simulink model "BimanualCarvingModifiedOldEMG"  (R2013a)
settings: Solver=ode4  SolverMode=SingleTasking  StartTime=0.0  StopTime=inf  FixedStep=0.0005  RelTol=1e-3
StartFcn:
  |  warndlg('Dexterit-E models cannot run under simulation. Please compile your model and run it from within Dexterit-E.');set_param(bdroot,'SimulationCommand','stop')
model workspace (MAT data in the model file):
  BKIN_STEP_TIME = 0.0005
  col_x = 1
  col_y = 2
  WIDTH = 3
  HEIGHT = 4
  TARGET_COL = 1
  LOAD = 2
  TRAJ_DURATION_COL = 3
  MAX_LOAD = 2
  FORCE_ON = 1
  HAND_RADIUS = 6
  REST_COL = 4
  TRAINING_COL = 5
  HAND_COLOR = 5
  TARGET_STROKE = 8
  TARGET_RADIUS = 9
  xMaxCursor = 15
  yMaxCursor = 16
  TARGET_COLOR = 7
  START_X = 10
  START_Y = 11
  STIFFNESS_MATERIAL = 3
  MATERIAL_MASS = 4
  MATERIAL_DAMPING = 5
  STIFFNESS_HANDS = 6
  MATERIAL_GOAL_COLOR = 12
  SCALE_VIBRATION = 7
  STONE_WIDTH = 6
  MATERIAL_DUCTILITY = 8
  TARG_COLOR = 1
  TEXT_COLOR = 13
  TEXTBOX_WIDTH = 14
  TEXTBOX_HEIGHT = 15
  ROTATION = 16
  LABEL_TEXT = 17
  LABEL_COLOR = 18
  LABEL_HEIGHT = 19
  ADVANCE_EMG_PLACEMENT = 2
  ADVANCE_EMG_MAX = 3
  EMG_ADVANCE_BUTTON = 1
  EMG_MVC_BUTTON = 2
  START_TRIAL = 3
  END_TRIAL = 4
  MUSC_NUM = 2
  HAND_DISTANCE = 3
  SYN_NUM = 4
undefined symbols (not defined in the file or in its folder): slselsubs
libraries: xpclib x9, simulink x6, General x3, KINARM_loads x2, Video x2, KINARM_IO x1, KINARM_EP_loads x1
(part 1 of 6)
CloseFcn:
  | rtwprivate ssgencode ModelCloseRequest b2lab2d
settings Model: ModifiedComment=chris -- Wed Feb 16 09:18:30 2005 -- Version 1.1384  ModifiedHistory=Feb 16/05 - Add error repeat, add offset ramp  ExtModeArmWhenConnect=off  ExtModeLogAll=off  BufferReuse=off  Creator=Chris Grebeldinger  LastModifiedBy=BKIN TECHNOLOGIES
settings DataIOCC: LimitDataPoints=off  SignalLoggingSaveFormat=ModelDataLogs  SaveOutput=off  SaveTime=off  SignalLoggingName=sigsOut
settings OptimizationCC: BlockReduction=off  BooleanDataType=off  OptimizeBlockIOStorage=off  BufferReuse=off  ExpressionFolding=off  ExpressionDepthLimit=2147483647  FoldNonRolledExpr=off  LocalBlockOutputs=off  InitFltsAndDblsToZero=on
settings DebuggingCC: SaveWithParameterizedLinksMsg=none  SignalResolutionControl=TryResolveAllWithWarning  SolverPrmCheckMsg=none  MultiTaskDSMMsg=warning  MultiTaskCondExecSysMsg=none  FcnCallInpInsideContextMsg=UseLocalSettings  StrictBusMsg=None
settings HardwareCC: ProdIntDivRoundTo=Zero  ProdEndianess=LittleEndian  ProdHWDeviceType=Generic->32-bit x86 compatible  TargetHWDeviceType=32-bit Generic
settings SFSimCC: SimParseCustomCode=off
settings RTWCC: SystemTargetFile=xpctarget.tlc  TemplateMakefile=xpc_default_tmf  Description=xPC Target  ProcessScript=xpctarget_make_rtw_hook  IncludeERTFirstTime=on  RTWCompilerOptimization=On
settings CodeAppCC: MaxIdLength=63
settings xpcTargetCC: TargetFcnLib=ansi_tfl_tmw.mat  CodeReplacementLibrary=XPC_BLAS  ParMdlRefBuildCompliant=on  ConcurrentExecutionCompliant=on  CombineSignalStateStructs=off  MATLABClassNameForMDSCustomization=xpcAperiodicCustomization  GRTInterface=on  GenerateAllocFcn=off  xPCTaskExecutionProfile=off  xPCRL32EventNumber=5000  xPCisDownloadable=off  xPCLoadParamSetFile=off  xPCConcurrentTasks=off  xPCEnableSFAnimation=off

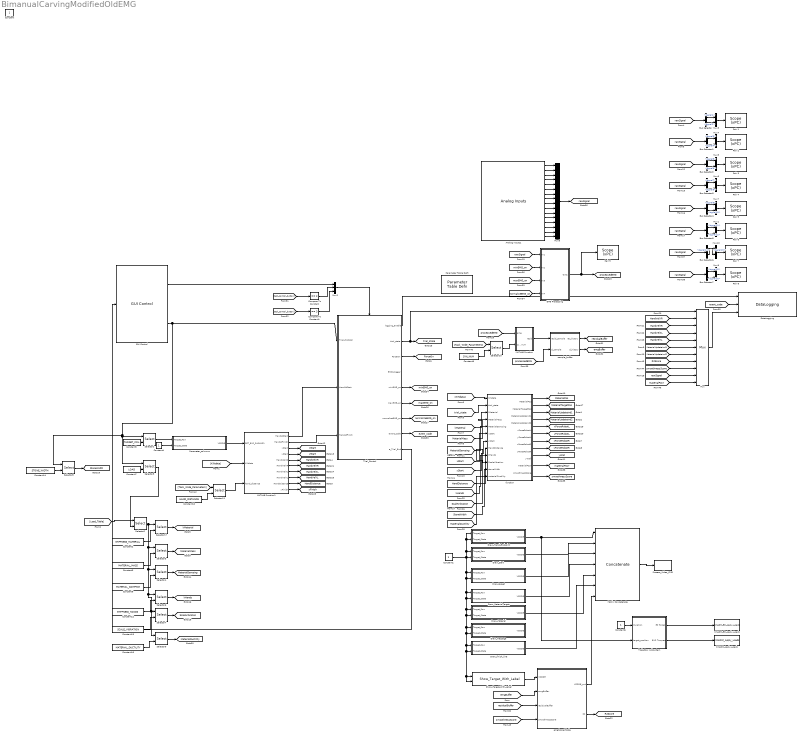
== system BimanualCarvingModifiedOldEMG ==
  Analog Inputs1 : KINARM_IO/Analog Inputs  channel=[1,2,3,4,5,6,7,8,9,10,11,12,13,14,15,16]  range=[5]  coupling=[0]  scantime6071e=1.28e-5  scantime6229=5e-6  sampletime=0.001  slot=-1  oscantime6071e=0
  Bus Selector : BusSelector  OutputSignals=signal1,signal2
  Bus Selector1 : BusSelector  OutputSignals=signal3,signal4
  Bus Selector2 : BusSelector  OutputSignals=signal5,signal6
  Bus Selector3 : BusSelector  OutputSignals=signal7,signal8
  Bus Selector4 : BusSelector  OutputSignals=signal9,signal10
  Bus Selector5 : BusSelector  OutputSignals=signal11,signal12
  Bus Selector6 : BusSelector  OutputSignals=signal13,signal14
  Bus Selector7 : BusSelector  OutputSignals=signal15,signal16
  Compare To Constant : simulink/Logic and Bit Operations/Compare To Constant  relop===  const=2  OutDataTypeStr=boolean
  Compare To Constant1 : simulink/Logic and Bit Operations/Compare To Constant  relop===  const=3  OutDataTypeStr=boolean
  Constant1 : Constant
  Constant10 : Constant  Value=HAND_DISTANCE
  Constant12 : Constant  Value=STIFFNESS_HANDS
  Constant13 : Constant  Value=SCALE_VIBRATION
  Constant14 : Constant  Value=STONE_WIDTH
  Constant16 : Constant  Value=MATERIAL_DUCTILITY
  Constant2 : Constant  Value=STIFFNESS_MATERIAL
  Constant3 : Constant  Value=MATERIAL_MASS
  Constant4 : Constant
  Constant5 : Constant  Value=TARGET_COL
  Constant6 : Constant
  Constant7 : Constant  Value=LOAD
  Constant8 : Constant  Value=MATERIAL_DAMPING
  Constant9 : Constant  Value=SYN_NUM
  DataLogging : General/DataLogging  log_event_codes=on  log_analog_inputs=on
      link override Poll KINARM/EPTorqueCMD: GotoTag=KINARMEPTorqueCMD
      link override Poll KINARM/TorqueCMD: GotoTag=KINARMTorqueCMD
      link override Poll KINARM/ZeroEPTorque: Value=[0 0 0 0]
      link override Poll KINARM/ZeroTorque: Value=[0 0 0 0]
  Draw_Hand_Endpoint : Subsystem  AncestorBlock=Video/Show_Target_With_Label  mask(Show_Target_With_Label){target_type=Circle, num_states=1, attribcol1=[HAND_COLOR HAND_COLOR HAND_RADIUS HAND_RADIUS 0 0 0], attribcol2=[6 6 0 3 0 0 0], attribcol3=[0 0 0 0 0 0 0], attribcol4=[0 0 0 0 0 0 0], attribcol5=[0 0 24 0 0 0 0], stateindices_padding=[0 0 0 0;0 0 0 0;0 0 0 0;0 0 0 0;0 0 0 0], source=dialog, opacity=100, target_display=Both subject and operator displays}
      mask prompts: target_type "Type of Target"; num_states "Number of Target States"; attribcol1 "State 1 Target Table Column(s)"; attribcol2 "State 2 Target Table Column(s)"; attribcol3 "State 3 Target Table Column(s)"; attribcol4 "State 4 Target Table Column(s)"; attribcol5 "State 5 Target Table Column(s)"; stateindices_padding "State Indices Padding"; source "Source for Opacity"; target_display "Target Display"
      mask help: This block returns a VCODE that, when sent to the Process_Video_CMD block, will cause a single target with a text label to be drawn. The label will be centered at the centroid of the target. Target parameters are specified in the Target Table according to the columns defined below and the row input to this block.
      mask init:
      | block_path = gcb;  % store block path, as gcb may change with block operations
      | 
      | %%% Get the model's workspace, because it is required to evaluate constants from the Parameter Table Def'n block
      | modelName=bdroot(block_path);
      | modelWorkspace = get_param(modelName, 'ModelWorkspace');
      | 
      | %%% Handle background colours if link status changes.  
      | checkBackgroundColour(block_path, 'Video');
      | 
      | %%% create the names of the input and output ports to display on the mask
      | output_block=char(find_system(block_path,'LookUnderMasks','all','FollowLinks','on','SearchDepth',1,'BlockType','Outport'));
      | outputname=get_param(output_block,'Name');
      | 
      | input_block=find_system(block_path,'LookUnderMasks','all','FollowLinks','on','SearchDepth',1,'BlockType','Inport');
      | inputname1=get_param(char(input_block{1}),'Name');
      | inputname2=get_param(char(input_block{2}),'Name');
      | if length(input_block) >= 3
      |     inputname3=get_param(char(input_block{3}),'Name');
      | end
      | 
      | %%%%%%%%%%%%%%%%%%%%%%%%%%%%%%%%%%%%%%%%%%%%%%%%%%%%%%%%%%%%%
      | %%% Create or replace the opacity input port
      | % Note: in earlier versions of MATLAB, the replace_block function did not work properly. When we drop support for R2007b,
      | % Check to see if it works properly in R2010a and if so, then this code can be simplified with the use of the replace_block function
      | sourceStr=get_param(block_path,'source');
      | 
      | if strmatch(sourceStr, 'dialog')
      | 	if length(input_block) == 3
      | 		pos=get_param([block_path '/Opacity'],'position');
      | 		delete_line(block_path, 'Opacity/1', 'Embedded MATLAB Function/4');
      | 		delete_block(input_block{3});
      |         add_block('built-in/Constant',[block_path '/Opacity'],'Name','Opacity');
      | 		set_param([block_path '/Opacity'],'position',pos);
      | 		add_line(block_path, 'Opacity/1', 'Embedded MATLAB Function/4');
      | 		set_param([block_path '/Opacity'],'Value','opacity');
      | 	end
      | 	displaytext = ['disp(columntext); port_label(''output'',1,outputname); port_label(''input'',1, inputname1); port_label(''input'',2, inputname2);'];
      | else
      | 	if length(input_block) == 2
      | 		pos=get_param([block_path '/Opacity'],'position');
      | 		delete_line(block_path, 'Opacity/1', 'Embedded MATLAB Function/4');
      | 		delete_block([block_path, '/Opacity']);
      | 		add_block('built-in/Inport',[block_path '/In2'],'Name','Opacity');
      | 		set_param([block_path '/Opacity'],'position',pos);
      | 		add_line(block_path, 'Opacity/1', 'Embedded MATLAB Function/4');
      |  	end
      | 	inputname3='Opacity';
      | 	displaytext = ['disp(columntext); port_label(''output'',1,outputname); port_label(''input'',1, inputname1); port_label(''input'',2, inputname2); port_label(''input'',3, inputname3);'];
      | end
      | set_param(block_path,'MaskDisplay',displaytext);
      | 
      | 
      | %%%%%%%%%%%%%%%%%%%%%%%%%%%%%%%%%%%%%%%%%%%%%%%%%%%%%%%%%%%%%
      | %%% Check and format the input strings for the vectors of column entires
      | targetTypeStr=get_param(block_path, 'target_type');
      | 
      | switch targetTypeStr(1:3)
      | 	case 'Cir',		numCol = 7;
      | 	case 'Ell',		numCol = 9;
      |     case 'Rec',		numCol = 9;
      |     case 'Lin',		numCol = 8;
      |     case 'Tri',		numCol = 10;
      | 	otherwise,		numCol = 7;
      | end
      | 
      | % % % numCol=str2num( get_param(block_path, 'num_col') );
      | for ii = 1:5
      | 	variableName = ['attribcol' num2str(ii)];
      | 	attribcoltext = get_param(block_path, variableName);
      | 	attribcoltext = checkUserInputVectorLength(attribcoltext, numCol);
      | 	set_param(block_path, variableName, attribcoltext);
      | end
      | 
      | % the input to the Embedded MATLAB script under the mask needs to have a certain size. This creates 'padding' to add to the 
      | % attribcol vectors to get to that size
      | zeros_5x7_matrix = zeros(5,7);
      | set_param(block_path, 'stateindices_padding', mat2str(zeros_5x7_matrix(:, 1:(11-numCol))) );
      | 
      | 
      | %%%%%%%%%%%%%%%%%%%%%%%%%%%%%%%%%%%%%%%%%%%%%%%%%%%%%%%%%%%%%
      | %%% Create the text to show on the mask
      | numStates = str2num(get_param(block_path, 'num_states'));
      | 
      | for ii = 1:numStates
      | 	variableName = ['attribcol' num2str(ii)];
      | 	attribcolString = get_param(block_path, variableName);
      | 	if isempty(modelWorkspace)
      | 		% if the block is part of a library, then modelWorkspace will be empty and the other code to evaluate attribcolStringEval will fail
      | 		attribcolStringEval = '[4 0 3 0 0 0 0]';
      | 	else
      | 		[attribcolValue, errorMessage] = BKINevalin(modelWorkspace, attribcolString);
      | 		attribcolStringEval = ['          ' mat2str( attribcolValue )];
      | 	end
      | 	if ii > 1
      | 		columntext = strvcat(columntext, attribcolStringEval);
      | 	else
      | 		columntext = attribcolStringEval;
      | 	end
      | end
      | 
      | % Add formatting spaces so that the mask looks nice
      | space = repmat(' ', 1, round(length(columntext)/2));
      | columntext=strvcat([space '(columns)'], columntext);
      mask Help:
      | Used to draw a single, stationary target with a label.
      | 
      | <H2>Library </H2>
      | Video
      | 
      | <H2>Description </H2>
      | This block returns a VCODE, which when sent to the Process_Video_CMD block will draw a single stationary target with a label. The VCODE contains all of the target parameters necessary to draw the target and the label.
      | <P>
      | The VCODE is generated from information contained in the Target Table. Which parts of the Target Table are used is determined by the columns selected (see Parameters and Dialog Box below).<P>
      | 
      | <p>For example, assume the "row" input is 2, the "type of target" is set to "rectangle" and the "Target Table Columns" is set to [3 0 0 4 5 0 6 7 4].
      | Then using the sample target table below a red rectangle will be drawn at (20cm, 40cm) with a width of 10cm and a height of 3cm.
      | The rectangle will have the word "Maybe" in yellow on it in letters 3cm heigh. The zeros in the  "Target Table Columns" indicate those parameters are not used (i.e. no stroke color, no stroke width, and no rotation).
      | 
      | <p><tt>
      | ______________________________________________________________________<br>
      | |&nbsp;&nbsp;&nbsp;&nbsp;&nbsp;&nbsp;&nbsp;&nbsp;&nbsp;&nbsp;| X Pos | Y pos |&nbsp;&nbsp;Fill | Width | Height |&nbsp;&nbsp;Text | TColor |<br>
      | ----------------------------------------------------------------------<br>
      | | target 1 |&nbsp;&nbsp;&nbsp;&nbsp;10 |&nbsp;&nbsp;&nbsp;&nbsp;10 | white |&nbsp;&nbsp;&nbsp;&nbsp;&nbsp;5 |&nbsp;&nbsp;&nbsp;&nbsp;&nbsp;&nbsp;2 |&nbsp;&nbsp;&nbsp;Yes |&nbsp;&nbsp;green |<br>
      | | target 2 |&nbsp;&nbsp;&nbsp;&nbsp;20 |&nbsp;&nbsp;&nbsp;&nbsp;40 |&nbsp;&nbsp;&nbsp;red |&nbsp;&nbsp;&nbsp;&nbsp;10 |&nbsp;&nbsp;&nbsp;&nbsp;&nbsp;&nbsp;3 | Maybe | yellow |<br>
      | | target 3 |&nbsp;&nbsp;&nbsp;-40 |&nbsp;&nbsp;&nbsp;&nbsp;10 |&nbsp;&nbsp;blue |&nbsp;&nbsp;&nbsp;&nbsp;&nbsp;3 |&nbsp;&nbsp;&nbsp;&nbsp;&nbsp;&nbsp;4 | Wrong |&nbsp;&nbsp;&nbsp;&nbsp;red |
      | ----------------------------------------------------------------------<br>
      | 
      | 
      | </tt>
      | 
      | 
      | <p>Inputs:<br>
      | <B> Target_Row: </B> this scalar input determines which row in the Target Table is used to define the target parameters. Typically the Target_Row comes from the Trial_Protocol.  <P>
      | <B> Target_State: </B> this scalar input determines which state the target is in. Different states reference different columns in the Target Table (as defined in the Dialog Box). Typically the Target_State input is controlled by the Stateflow chart to dynamically change the appearance of the target depending on system and/or subject behavior. Target_State=0 is a valid input, which turns the target off. The intended method for turning a target off is to set Target_State=0. <BR>
      | <P>
      | <B>Opacity:</B> This input is only available if Source for Opacity is selected as port, in which case the opacity for all of the targets created by this block is specified as a percentage.
      | The length of this input must either match the length of the Target_Row(s) input (i.e. which case each Opacity maps to the appropriate Target_row)
      | or this input must be a scalar (in which case the Opacity maps to all of the Target_Rows).<BR>
      | <P>
      | There is one output from this block:
      | <P>
      | <B> VCODE: </B> this output is a vector containing one VCODE. This output must go to the Process_Video_CMD block of the video library for the target to actually be shown (if any other visual targets are to be displayed, then this VCODE output must be concatenated with the other VCODES prior to connection to the Process_Video_CMD block - see Help for the Process_Video_CMD block for more information).
      | <P>
      | To show multiple targets simultaneously, multiple copies of the Show_Target and Show_Target_With_Label blocks can be used in a Task Program. The output VCODES from multiple Show_Target and Show_Target_With_Label blocks must be concatenated prior to connection to the Process_Video_CMD block.
      | <P>
      | 
      | <H2>Parameters and Dialog Box</H2>
      | <B>Type of Target:</B> Choose the type of target specified in the target table.
      | <P>
      | <B>Number of Target States:</B> Choose the number of target states specified in each target row. Up to five target states are allowed per target row.
      | <P>
      | <B>State [n] Target Table Columns:</B> Enter the column indices that specify the relevant target attributes in the Target Table. All target types have the same first three target attributes (fill colour, stroke colour and stroke width) and the same last three target attributes (label text, label colour, and label height).
      | <Blockquote>
      | <P>
      | Element 1 (fill colour) - points to the column index in the Target Table containing the fill colour. If this index is 0, then the fill colour is transparent and the Target Table is not referenced. For line targets, the fill colour is not used.
      | <P>
      | Element 2 (stroke colour) - points to the column index in the Target Table containing the stroke colour. If this index is 0, then the stroke colour is transparent and the Target Table is not referenced. It is possible to use the same column index for both fill colour and stroke colour (i.e.  if single-colour targets are desired). For line targets, stroke colour defines the colour of the line.
      | <P>
      | Element 3 (stroke width) - points to the column index in the Target Table containing the stroke width (cm). If no stroke is desired, then setting the stroke column index to 0 will produce a stroke width of 0  and the Target Table is not referenced.  Setting stroke column index to a value less than 0 will produce a standard 1 mm stroke width, again without referencing the Target Table. For line targets, stroke width defines the width of the line.
      | <P>
      | <B><I>Circle</I></B> <P>
      | Element 4 (radius) - radius of the circle (cm).
      | <P>
      | <B><I>Ellipse</I></B> <P>
      | Elements 4-6 (ellipse properties) - major radius (cm), minor radius (cm), rotation angle (degrees). If no rotation is desired, then setting rotation column index to 0 will produce a default rotation of 0 and the Target Table will not be referenced.
      | <P>
      | <B><I>Rectangle</I></B><P>
      | Elements 4-6 (rectangle properties) - length (cm), height (cm), rotation angle (degrees). If no rotation is desired, then setting rotation column index to 0 will produce a default rotation of 0 and the Target Table will not be referenced.
      | <P>
      | <B><I>Line</I></B><P>
      | Elements 4-5 (line properties) - end point x-axis position relative to start point (cm), end point y-axis position relative to start point (cm). The width and colour of the line are defined by the stroke width and the stroke colour, respectively. The fill colour column is ignored (i.e. any value can be used for column 1)
      | <P>
      | <B><I>Triangle</I></B><P>
      | Elements 4-7 (triangle properties) - length (cm), height (cm), offset of peak of triangle relative to midpoint of the length (cm), rotation angle (degrees). If a height column index of 0 is specified, then an equilateral triangle with sides of the specified length will be created and the Target Table will not be referenced for height or peak offset. If no rotation is desired, then setting a rotation column index of 0 will produce a default rotation of 0 and the Target Table will not be referenced.
      | <P>
      | <B><I>Label</I></B>
      | <P>
      | The last three elements of the target state vector define the label. In order, these elements are:
      | <P>
      | Label text - the index of the column in the Target Table containing the text used for the label (up to 50 characters).
      | <P>
      | Label colour - the index of the column in the Target Table containing the label colour. If this index is 0, then the label colour is transparent and the Target Table is not referenced.
      | <P>
      | Label height - the index of the column in the Target Table containing the label height (cm).
      | </Blockquote>
      | <P>
      | Each target state requires its own set of column index definitions (although multiple states can point to the same column index if desired).<P>
      | 
      | <B>Source for Opacity:</B> Choose either dialog, to specify the opacity in this dialog, or port, which will create a new input to allow dynamic control of opacity.
      | <P>
      | <B>Opacity:</B> This parameter is only available if Source for Opacity is selected as dialog, in which case the opacity for all of the targets created by this block is specified as a percentage.
      | <P>
      | <B>Target Display:</B> This option determines whether the target(s) are shown on the operator display only, the subject display only, or both displays.
      | <P>
      | 
      | <H2>Examples</H2>
      | 
      | <B>Example 1:</B>  Suppose a target row will be used to define 1 state for an ellipse type target. It will be an outline of an ellipse with a label in the center (using a stroke colour and a standard 1mm stroke width). The related Target Table columns are:
      | <P>
      | column 4 = colour<BR>
      | column 5 = major radius<BR>
      | column 6 = minor radius<BR>
      | column 7 = orientation<BR>
      | column 8 = label text<BR>
      | column 9 = label colour<BR>
      | column 10 = label height
      | <P>For this example, "State 1 Target Table Columns" would equal [0 4 -1 5 6 7 8 9 10].
      | <P>
      | 
      | <H2>Related Blocks </H2>
      | Show_Target<BR>
      | Process_Video_CMD
      mask TypeOptions target_type: Circle | Ellipse | Rectangle | Line | Triangle
      mask Callback target_type:
      | %%%%
      | % Because of bugs iN R2007, R2010a and R2013a (which have been reported to Mathworks), the following code
      | % is required here because in the Initialization Section it will ONLY correctly update those Mask Parameters that are hidden
      | % when the OK button is clicked (NOTE: the initialization code will correctly update all Mask Parameters when the Apply button
      | % is clicked, the bug is that it should also update everything when the OK button is clicked in the absence of an Apply click)
      | %
      | % Adding a set_param call which updates one of the mask parameters will call the initialization code to run, which "avoids"
      | % this bug. This code should be removed once Mathworks has fixed this bug.
      | 
      | temp = get_param(gcb, 'target_type');
      | set_param(gcb, 'target_type', temp);
      mask TypeOptions num_states: 1 | 2 | 3 | 4 | 5
      mask Callback num_states:
      | block_path=gcb;
      | num_states=str2num(get_param(block_path, 'num_states'));
      | vis=get_param(block_path,'MaskVisibilities');
      | 
      | %If the number of states>1, then output an array instead of a vector.
      | %Only show those inputs necessary on the Mask
      | output_block=char(find_system(block_path,'LookUnderMasks','all','SearchDepth',1,'BlockType','Outport'));
      | if num_states==1			%output of HandInTarget block is a vector
      | 	vis{4}='off';
      | 	vis{5}='off';
      | 	vis{6}='off';
      | 	vis{7}='off';
      | elseif num_states==2					%output of HandInTarget block is an array
      | 	vis{4}='on';
      | 	vis{5}='off';
      | 	vis{6}='off';
      | 	vis{7}='off';
      | elseif num_states==3					%output of HandInTarget block is an array
      | 	vis{4}='on';
      | 	vis{5}='on';
      | 	vis{6}='off';
      | 	vis{7}='off';
      | elseif num_states==4					%output of HandInTarget block is an array
      | 	vis{4}='on';
      | 	vis{5}='on';
      | 	vis{6}='on';
      | 	vis{7}='off';
      | else								%output of HandInTarget block is an array
      | 	vis{4}='on';
      | 	vis{5}='on';
      | 	vis{6}='on';
      | 	vis{7}='on';
      | end
      | set_param(block_path,'MaskVisibilities',vis);
      mask TypeOptions source: dialog | port
      mask Callback source:
      | % Show or hide the opacity input on the mask dialog
      | sourceStr=get_param(gcb,'source');
      | vis=get_param(gcb,'MaskVisibilities');
      | 
      | if strmatch(sourceStr, 'dialog')
      | 	vis{10}='on';
      | else
      | 	vis{10}='off';
      | end
      | 
      | set_param(gcb,'MaskVisibilities',vis);
      mask TypeOptions target_display: Both subject and operator displays | Subject display only | Operator display only
      mask Display: disp(columntext); port_label('output',1,outputname); port_label('input',1, inputname1); port_label('input',2, inputname2);
  Draw_Material : Subsystem  AncestorBlock=Video/Show_Target_With_Label  mask(Show_Target_With_Label){target_type=Line, num_states=1, attribcol1=[TARGET_COLOR TARGET_COLOR TARGET_STROKE TARGET_RADIUS 0 0 0 0], attribcol2=[6 6 0 3 0 0 0 0], attribcol3=[0 0 0 0 0 0 0 0], attribcol4=[0 0 0 0 0 0 0 0], attribcol5=[0 0 24 0 0 0 0 0], stateindices_padding=[0 0 0;0 0 0;0 0 0;0 0 0;0 0 0], source=dialog, opacity=100, target_display=Both subject and operator displays}
      mask prompts: target_type "Type of Target"; num_states "Number of Target States"; attribcol1 "State 1 Target Table Column(s)"; attribcol2 "State 2 Target Table Column(s)"; attribcol3 "State 3 Target Table Column(s)"; attribcol4 "State 4 Target Table Column(s)"; attribcol5 "State 5 Target Table Column(s)"; stateindices_padding "State Indices Padding"; source "Source for Opacity"; target_display "Target Display"
      mask help: This block returns a VCODE that, when sent to the Process_Video_CMD block, will cause a single target with a text label to be drawn. The label will be centered at the centroid of the target. Target parameters are specified in the Target Table according to the columns defined below and the row input to this block.
      mask init: same as BimanualCarvingModifiedOldEMG/Draw_Hand_Endpoint
      mask Help:
      | Used to draw a single, stationary target with a label.
      | 
      | <H2>Library </H2>
      | Video
      | 
      | <H2>Description </H2>
      | This block returns a VCODE, which when sent to the Process_Video_CMD block will draw a single stationary target with a label. The VCODE contains all of the target parameters necessary to draw the target and the label.
      | <P>
      | The VCODE is generated from information contained in the Target Table. Which parts of the Target Table are used is determined by the columns selected (see Parameters and Dialog Box below).<P>
      | 
      | <p>For example, assume the "row" input is 2, the "type of target" is set to "rectangle" and the "Target Table Columns" is set to [3 0 0 4 5 0 6 7 4].
      | Then using the sample target table below a red rectangle will be drawn at (20cm, 40cm) with a width of 10cm and a height of 3cm.
      | The rectangle will have the word "Maybe" in yellow on it in letters 3cm heigh. The zeros in the  "Target Table Columns" indicate those parameters are not used (i.e. no stroke color, no stroke width, and no rotation).
      | 
      | <p><tt>
      | ______________________________________________________________________<br>
      | |&nbsp;&nbsp;&nbsp;&nbsp;&nbsp;&nbsp;&nbsp;&nbsp;&nbsp;&nbsp;| X Pos | Y pos |&nbsp;&nbsp;Fill | Width | Height |&nbsp;&nbsp;Text | TColor |<br>
      | ----------------------------------------------------------------------<br>
      | | target 1 |&nbsp;&nbsp;&nbsp;&nbsp;10 |&nbsp;&nbsp;&nbsp;&nbsp;10 | white |&nbsp;&nbsp;&nbsp;&nbsp;&nbsp;5 |&nbsp;&nbsp;&nbsp;&nbsp;&nbsp;&nbsp;2 |&nbsp;&nbsp;&nbsp;Yes |&nbsp;&nbsp;green |<br>
      | | target 2 |&nbsp;&nbsp;&nbsp;&nbsp;20 |&nbsp;&nbsp;&nbsp;&nbsp;40 |&nbsp;&nbsp;&nbsp;red |&nbsp;&nbsp;&nbsp;&nbsp;10 |&nbsp;&nbsp;&nbsp;&nbsp;&nbsp;&nbsp;3 | Maybe | yellow |<br>
      | | target 3 |&nbsp;&nbsp;&nbsp;-40 |&nbsp;&nbsp;&nbsp;&nbsp;10 |&nbsp;&nbsp;blue |&nbsp;&nbsp;&nbsp;&nbsp;&nbsp;3 |&nbsp;&nbsp;&nbsp;&nbsp;&nbsp;&nbsp;4 | Wrong |&nbsp;&nbsp;&nbsp;&nbsp;red |
      | ----------------------------------------------------------------------<br>
      | 
      | 
      | </tt>
      | 
      | 
      | <p>Inputs:<br>
      | <B> Target_Row: </B> this scalar input determines which row in the Target Table is used to define the target parameters. Typically the Target_Row comes from the Trial_Protocol.  <P>
      | <B> Target_State: </B> this scalar input determines which state the target is in. Different states reference different columns in the Target Table (as defined in the Dialog Box). Typically the Target_State input is controlled by the Stateflow chart to dynamically change the appearance of the target depending on system and/or subject behavior. Target_State=0 is a valid input, which turns the target off. The intended method for turning a target off is to set Target_State=0. <BR>
      | <P>
      | <B>Opacity:</B> This input is only available if Source for Opacity is selected as port, in which case the opacity for all of the targets created by this block is specified as a percentage.
      | The length of this input must either match the length of the Target_Row(s) input (i.e. which case each Opacity maps to the appropriate Target_row)
      | or this input must be a scalar (in which case the Opacity maps to all of the Target_Rows).<BR>
      | <P>
      | There is one output from this block:
      | <P>
      | <B> VCODE: </B> this output is a vector containing one VCODE. This output must go to the Process_Video_CMD block of the video library for the target to actually be shown (if any other visual targets are to be displayed, then this VCODE output must be concatenated with the other VCODES prior to connection to the Process_Video_CMD block - see Help for the Process_Video_CMD block for more information).
      | <P>
      | To show multiple targets simultaneously, multiple copies of the Show_Target and Show_Target_With_Label blocks can be used in a Task Program. The output VCODES from multiple Show_Target and Show_Target_With_Label blocks must be concatenated prior to connection to the Process_Video_CMD block.
      | <P>
      | 
      | <H2>Parameters and Dialog Box</H2>
      | <B>Type of Target:</B> Choose the type of target specified in the target table.
      | <P>
      | <B>Number of Target States:</B> Choose the number of target states specified in each target row. Up to five target states are allowed per target row.
      | <P>
      | <B>State [n] Target Table Columns:</B> Enter the column indices that specify the relevant target attributes in the Target Table. All target types have the same first three target attributes (fill colour, stroke colour and stroke width) and the same last three target attributes (label text, label colour, and label height).
      | <Blockquote>
      | <P>
      | Element 1 (fill colour) - points to the column index in the Target Table containing the fill colour. If this index is 0, then the fill colour is transparent and the Target Table is not referenced. For line targets, the fill colour is not used.
      | <P>
      | Element 2 (stroke colour) - points to the column index in the Target Table containing the stroke colour. If this index is 0, then the stroke colour is transparent and the Target Table is not referenced. It is possible to use the same column index for both fill colour and stroke colour (i.e.  if single-colour targets are desired). For line targets, stroke colour defines the colour of the line.
      | <P>
      | Element 3 (stroke width) - points to the column index in the Target Table containing the stroke width (cm). If no stroke is desired, then setting the stroke column index to 0 will produce a stroke width of 0  and the Target Table is not referenced.  Setting stroke column index to a value less than 0 will produce a standard 1 mm stroke width, again without referencing the Target Table. For line targets, stroke width defines the width of the line.
      | <P>
      | <B><I>Circle</I></B> <P>
      | Element 4 (radius) - radius of the circle (cm).
      | <P>
      | <B><I>Ellipse</I></B> <P>
      | Elements 4-6 (ellipse properties) - major radius (cm), minor radius (cm), rotation angle (degrees). If no rotation is desired, then setting rotation column index to 0 will produce a default rotation of 0 and the Target Table will not be referenced.
      | <P>
      | <B><I>Rectangle</I></B><P>
      | Elements 4-6 (rectangle properties) - length (cm), height (cm), rotation angle (degrees). If no rotation is desired, then setting rotation column index to 0 will produce a default rotation of 0 and the Target Table will not be referenced.
      | <P>
      | <B><I>Line</I></B><P>
      | Elements 4-5 (line properties) - end point x-axis position relative to start point (cm), end point y-axis position relative to start point (cm). The width and colour of the line are defined by the stroke width and the stroke colour, respectively. The fill colour column is ignored (i.e. any value can be used for column 1)
      | <P>
      | <B><I>Triangle</I></B><P>
      | Elements 4-7 (triangle properties) - length (cm), height (cm), offset of peak of triangle relative to midpoint of the length (cm), rotation angle (degrees). If a height column index of 0 is specified, then an equilateral triangle with sides of the specified length will be created and the Target Table will not be referenced for height or peak offset. If no rotation is desired, then setting a rotation column index of 0 will produce a default rotation of 0 and the Target Table will not be referenced.
      | <P>
      | <B><I>Label</I></B>
      | <P>
      | The last three elements of the target state vector define the label. In order, these elements are:
      | <P>
      | Label text - the index of the column in the Target Table containing the text used for the label (up to 50 characters).
      | <P>
      | Label colour - the index of the column in the Target Table containing the label colour. If this index is 0, then the label colour is transparent and the Target Table is not referenced.
      | <P>
      | Label height - the index of the column in the Target Table containing the label height (cm).
      | </Blockquote>
      | <P>
      | Each target state requires its own set of column index definitions (although multiple states can point to the same column index if desired).<P>
      | 
      | <B>Source for Opacity:</B> Choose either dialog, to specify the opacity in this dialog, or port, which will create a new input to allow dynamic control of opacity.
      | <P>
      | <B>Opacity:</B> This parameter is only available if Source for Opacity is selected as dialog, in which case the opacity for all of the targets created by this block is specified as a percentage.
      | <P>
      | <B>Target Display:</B> This option determines whether the target(s) are shown on the operator display only, the subject display only, or both displays.
      | <P>
      | 
      | <H2>Examples</H2>
      | 
      | <B>Example 1:</B>  Suppose a target row will be used to define 1 state for an ellipse type target. It will be an outline of an ellipse with a label in the center (using a stroke colour and a standard 1mm stroke width). The related Target Table columns are:
      | <P>
      | column 4 = colour<BR>
      | column 5 = major radius<BR>
      | column 6 = minor radius<BR>
      | column 7 = orientation<BR>
      | column 8 = label text<BR>
      | column 9 = label colour<BR>
      | column 10 = label height
      | <P>For this example, "State 1 Target Table Columns" would equal [0 4 -1 5 6 7 8 9 10].
      | <P>
      | 
      | <H2>Related Blocks </H2>
      | Show_Target<BR>
      | Process_Video_CMD
      mask TypeOptions target_type: Circle | Ellipse | Rectangle | Line | Triangle
      mask Callback target_type:
      | %%%%
      | % Because of bugs iN R2007, R2010a and R2013a (which have been reported to Mathworks), the following code
      | % is required here because in the Initialization Section it will ONLY correctly update those Mask Parameters that are hidden
      | % when the OK button is clicked (NOTE: the initialization code will correctly update all Mask Parameters when the Apply button
      | % is clicked, the bug is that it should also update everything when the OK button is clicked in the absence of an Apply click)
      | %
      | % Adding a set_param call which updates one of the mask parameters will call the initialization code to run, which "avoids"
      | % this bug. This code should be removed once Mathworks has fixed this bug.
      | 
      | temp = get_param(gcb, 'target_type');
      | set_param(gcb, 'target_type', temp);
      mask TypeOptions num_states: 1 | 2 | 3 | 4 | 5
      mask Callback num_states:
      | block_path=gcb;
      | num_states=str2num(get_param(block_path, 'num_states'));
      | vis=get_param(block_path,'MaskVisibilities');
      | 
      | %If the number of states>1, then output an array instead of a vector.
      | %Only show those inputs necessary on the Mask
      | output_block=char(find_system(block_path,'LookUnderMasks','all','SearchDepth',1,'BlockType','Outport'));
      | if num_states==1			%output of HandInTarget block is a vector
      | 	vis{4}='off';
      | 	vis{5}='off';
      | 	vis{6}='off';
      | 	vis{7}='off';
      | elseif num_states==2					%output of HandInTarget block is an array
      | 	vis{4}='on';
      | 	vis{5}='off';
      | 	vis{6}='off';
      | 	vis{7}='off';
      | elseif num_states==3					%output of HandInTarget block is an array
      | 	vis{4}='on';
      | 	vis{5}='on';
      | 	vis{6}='off';
      | 	vis{7}='off';
      | elseif num_states==4					%output of HandInTarget block is an array
      | 	vis{4}='on';
      | 	vis{5}='on';
      | 	vis{6}='on';
      | 	vis{7}='off';
      | else								%output of HandInTarget block is an array
      | 	vis{4}='on';
      | 	vis{5}='on';
      | 	vis{6}='on';
      | 	vis{7}='on';
      | end
      | set_param(block_path,'MaskVisibilities',vis);
      mask TypeOptions source: dialog | port
      mask Callback source:
      | % Show or hide the opacity input on the mask dialog
      | sourceStr=get_param(gcb,'source');
      | vis=get_param(gcb,'MaskVisibilities');
      | 
      | if strmatch(sourceStr, 'dialog')
      | 	vis{10}='on';
      | else
      | 	vis{10}='off';
      | end
      | 
      | set_param(gcb,'MaskVisibilities',vis);
      mask TypeOptions target_display: Both subject and operator displays | Subject display only | Operator display only
      mask Display: disp(columntext); port_label('output',1,outputname); port_label('input',1, inputname1); port_label('input',2, inputname2);
  Draw_MaterialTarget : Subsystem  AncestorBlock=Video/Show_Target_With_Label  mask(Show_Target_With_Label){target_type=Line, num_states=1, attribcol1=[MATERIAL_GOAL_COLOR MATERIAL_GOAL_COLOR TARGET_STROKE TARGET_RADIUS 0 0 0 0], attribcol2=[6 6 0 3 0 0 0 0], attribcol3=[0 0 0 0 0 0 0 0], attribcol4=[0 0 0 0 0 0 0 0], attribcol5=[0 0 24 0 0 0 0 0], stateindices_padding=[0 0 0;0 0 0;0 0 0;0 0 0;0 0 0], source=dialog, opacity=100, target_display=Both subject and operator displays}
      mask prompts: target_type "Type of Target"; num_states "Number of Target States"; attribcol1 "State 1 Target Table Column(s)"; attribcol2 "State 2 Target Table Column(s)"; attribcol3 "State 3 Target Table Column(s)"; attribcol4 "State 4 Target Table Column(s)"; attribcol5 "State 5 Target Table Column(s)"; stateindices_padding "State Indices Padding"; source "Source for Opacity"; target_display "Target Display"
      mask help: This block returns a VCODE that, when sent to the Process_Video_CMD block, will cause a single target with a text label to be drawn. The label will be centered at the centroid of the target. Target parameters are specified in the Target Table according to the columns defined below and the row input to this block.
      mask init: same as BimanualCarvingModifiedOldEMG/Draw_Hand_Endpoint
      mask Help:
      | Used to draw a single, stationary target with a label.
      | 
      | <H2>Library </H2>
      | Video
      | 
      | <H2>Description </H2>
      | This block returns a VCODE, which when sent to the Process_Video_CMD block will draw a single stationary target with a label. The VCODE contains all of the target parameters necessary to draw the target and the label.
      | <P>
      | The VCODE is generated from information contained in the Target Table. Which parts of the Target Table are used is determined by the columns selected (see Parameters and Dialog Box below).<P>
      | 
      | <p>For example, assume the "row" input is 2, the "type of target" is set to "rectangle" and the "Target Table Columns" is set to [3 0 0 4 5 0 6 7 4].
      | Then using the sample target table below a red rectangle will be drawn at (20cm, 40cm) with a width of 10cm and a height of 3cm.
      | The rectangle will have the word "Maybe" in yellow on it in letters 3cm heigh. The zeros in the  "Target Table Columns" indicate those parameters are not used (i.e. no stroke color, no stroke width, and no rotation).
      | 
      | <p><tt>
      | ______________________________________________________________________<br>
      | |&nbsp;&nbsp;&nbsp;&nbsp;&nbsp;&nbsp;&nbsp;&nbsp;&nbsp;&nbsp;| X Pos | Y pos |&nbsp;&nbsp;Fill | Width | Height |&nbsp;&nbsp;Text | TColor |<br>
      | ----------------------------------------------------------------------<br>
      | | target 1 |&nbsp;&nbsp;&nbsp;&nbsp;10 |&nbsp;&nbsp;&nbsp;&nbsp;10 | white |&nbsp;&nbsp;&nbsp;&nbsp;&nbsp;5 |&nbsp;&nbsp;&nbsp;&nbsp;&nbsp;&nbsp;2 |&nbsp;&nbsp;&nbsp;Yes |&nbsp;&nbsp;green |<br>
      | | target 2 |&nbsp;&nbsp;&nbsp;&nbsp;20 |&nbsp;&nbsp;&nbsp;&nbsp;40 |&nbsp;&nbsp;&nbsp;red |&nbsp;&nbsp;&nbsp;&nbsp;10 |&nbsp;&nbsp;&nbsp;&nbsp;&nbsp;&nbsp;3 | Maybe | yellow |<br>
      | | target 3 |&nbsp;&nbsp;&nbsp;-40 |&nbsp;&nbsp;&nbsp;&nbsp;10 |&nbsp;&nbsp;blue |&nbsp;&nbsp;&nbsp;&nbsp;&nbsp;3 |&nbsp;&nbsp;&nbsp;&nbsp;&nbsp;&nbsp;4 | Wrong |&nbsp;&nbsp;&nbsp;&nbsp;red |
      | ----------------------------------------------------------------------<br>
      | 
      | 
      | </tt>
      | 
      | 
      | <p>Inputs:<br>
      | <B> Target_Row: </B> this scalar input determines which row in the Target Table is used to define the target parameters. Typically the Target_Row comes from the Trial_Protocol.  <P>
      | <B> Target_State: </B> this scalar input determines which state the target is in. Different states reference different columns in the Target Table (as defined in the Dialog Box). Typically the Target_State input is controlled by the Stateflow chart to dynamically change the appearance of the target depending on system and/or subject behavior. Target_State=0 is a valid input, which turns the target off. The intended method for turning a target off is to set Target_State=0. <BR>
      | <P>
      | <B>Opacity:</B> This input is only available if Source for Opacity is selected as port, in which case the opacity for all of the targets created by this block is specified as a percentage.
      | The length of this input must either match the length of the Target_Row(s) input (i.e. which case each Opacity maps to the appropriate Target_row)
      | or this input must be a scalar (in which case the Opacity maps to all of the Target_Rows).<BR>
      | <P>
      | There is one output from this block:
      | <P>
      | <B> VCODE: </B> this output is a vector containing one VCODE. This output must go to the Process_Video_CMD block of the video library for the target to actually be shown (if any other visual targets are to be displayed, then this VCODE output must be concatenated with the other VCODES prior to connection to the Process_Video_CMD block - see Help for the Process_Video_CMD block for more information).
      | <P>
      | To show multiple targets simultaneously, multiple copies of the Show_Target and Show_Target_With_Label blocks can be used in a Task Program. The output VCODES from multiple Show_Target and Show_Target_With_Label blocks must be concatenated prior to connection to the Process_Video_CMD block.
      | <P>
      | 
      | <H2>Parameters and Dialog Box</H2>
      | <B>Type of Target:</B> Choose the type of target specified in the target table.
      | <P>
      | <B>Number of Target States:</B> Choose the number of target states specified in each target row. Up to five target states are allowed per target row.
      | <P>
      | <B>State [n] Target Table Columns:</B> Enter the column indices that specify the relevant target attributes in the Target Table. All target types have the same first three target attributes (fill colour, stroke colour and stroke width) and the same last three target attributes (label text, label colour, and label height).
      | <Blockquote>
      | <P>
      | Element 1 (fill colour) - points to the column index in the Target Table containing the fill colour. If this index is 0, then the fill colour is transparent and the Target Table is not referenced. For line targets, the fill colour is not used.
      | <P>
      | Element 2 (stroke colour) - points to the column index in the Target Table containing the stroke colour. If this index is 0, then the stroke colour is transparent and the Target Table is not referenced. It is possible to use the same column index for both fill colour and stroke colour (i.e.  if single-colour targets are desired). For line targets, stroke colour defines the colour of the line.
      | <P>
      | Element 3 (stroke width) - points to the column index in the Target Table containing the stroke width (cm). If no stroke is desired, then setting the stroke column index to 0 will produce a stroke width of 0  and the Target Table is not referenced.  Setting stroke column index to a value less than 0 will produce a standard 1 mm stroke width, again without referencing the Target Table. For line targets, stroke width defines the width of the line.
      | <P>
      | <B><I>Circle</I></B> <P>
      | Element 4 (radius) - radius of the circle (cm).
      | <P>
      | <B><I>Ellipse</I></B> <P>
      | Elements 4-6 (ellipse properties) - major radius (cm), minor radius (cm), rotation angle (degrees). If no rotation is desired, then setting rotation column index to 0 will produce a default rotation of 0 and the Target Table will not be referenced.
      | <P>
      | <B><I>Rectangle</I></B><P>
      | Elements 4-6 (rectangle properties) - length (cm), height (cm), rotation angle (degrees). If no rotation is desired, then setting rotation column index to 0 will produce a default rotation of 0 and the Target Table will not be referenced.
      | <P>
      | <B><I>Line</I></B><P>
      | Elements 4-5 (line properties) - end point x-axis position relative to start point (cm), end point y-axis position relative to start point (cm). The width and colour of the line are defined by the stroke width and the stroke colour, respectively. The fill colour column is ignored (i.e. any value can be used for column 1)
      | <P>
      | <B><I>Triangle</I></B><P>
      | Elements 4-7 (triangle properties) - length (cm), height (cm), offset of peak of triangle relative to midpoint of the length (cm), rotation angle (degrees). If a height column index of 0 is specified, then an equilateral triangle with sides of the specified length will be created and the Target Table will not be referenced for height or peak offset. If no rotation is desired, then setting a rotation column index of 0 will produce a default rotation of 0 and the Target Table will not be referenced.
      | <P>
      | <B><I>Label</I></B>
      | <P>
      | The last three elements of the target state vector define the label. In order, these elements are:
      | <P>
      | Label text - the index of the column in the Target Table containing the text used for the label (up to 50 characters).
      | <P>
      | Label colour - the index of the column in the Target Table containing the label colour. If this index is 0, then the label colour is transparent and the Target Table is not referenced.
      | <P>
      | Label height - the index of the column in the Target Table containing the label height (cm).
      | </Blockquote>
      | <P>
      | Each target state requires its own set of column index definitions (although multiple states can point to the same column index if desired).<P>
      | 
      | <B>Source for Opacity:</B> Choose either dialog, to specify the opacity in this dialog, or port, which will create a new input to allow dynamic control of opacity.
      | <P>
      | <B>Opacity:</B> This parameter is only available if Source for Opacity is selected as dialog, in which case the opacity for all of the targets created by this block is specified as a percentage.
      | <P>
      | <B>Target Display:</B> This option determines whether the target(s) are shown on the operator display only, the subject display only, or both displays.
      | <P>
      | 
      | <H2>Examples</H2>
      | 
      | <B>Example 1:</B>  Suppose a target row will be used to define 1 state for an ellipse type target. It will be an outline of an ellipse with a label in the center (using a stroke colour and a standard 1mm stroke width). The related Target Table columns are:
      | <P>
      | column 4 = colour<BR>
      | column 5 = major radius<BR>
      | column 6 = minor radius<BR>
      | column 7 = orientation<BR>
      | column 8 = label text<BR>
      | column 9 = label colour<BR>
      | column 10 = label height
      | <P>For this example, "State 1 Target Table Columns" would equal [0 4 -1 5 6 7 8 9 10].
      | <P>
      | 
      | <H2>Related Blocks </H2>
      | Show_Target<BR>
      | Process_Video_CMD
      mask TypeOptions target_type: Circle | Ellipse | Rectangle | Line | Triangle
      mask Callback target_type:
      | %%%%
      | % Because of bugs iN R2007, R2010a and R2013a (which have been reported to Mathworks), the following code
      | % is required here because in the Initialization Section it will ONLY correctly update those Mask Parameters that are hidden
      | % when the OK button is clicked (NOTE: the initialization code will correctly update all Mask Parameters when the Apply button
      | % is clicked, the bug is that it should also update everything when the OK button is clicked in the absence of an Apply click)
      | %
      | % Adding a set_param call which updates one of the mask parameters will call the initialization code to run, which "avoids"
      | % this bug. This code should be removed once Mathworks has fixed this bug.
      | 
      | temp = get_param(gcb, 'target_type');
      | set_param(gcb, 'target_type', temp);
      mask TypeOptions num_states: 1 | 2 | 3 | 4 | 5
      mask Callback num_states:
      | block_path=gcb;
      | num_states=str2num(get_param(block_path, 'num_states'));
      | vis=get_param(block_path,'MaskVisibilities');
      | 
      | %If the number of states>1, then output an array instead of a vector.
      | %Only show those inputs necessary on the Mask
      | output_block=char(find_system(block_path,'LookUnderMasks','all','SearchDepth',1,'BlockType','Outport'));
      | if num_states==1			%output of HandInTarget block is a vector
      | 	vis{4}='off';
      | 	vis{5}='off';
      | 	vis{6}='off';
      | 	vis{7}='off';
      | elseif num_states==2					%output of HandInTarget block is an array
      | 	vis{4}='on';
      | 	vis{5}='off';
      | 	vis{6}='off';
      | 	vis{7}='off';
      | elseif num_states==3					%output of HandInTarget block is an array
      | 	vis{4}='on';
      | 	vis{5}='on';
      | 	vis{6}='off';
      | 	vis{7}='off';
      | elseif num_states==4					%output of HandInTarget block is an array
      | 	vis{4}='on';
      | 	vis{5}='on';
      | 	vis{6}='on';
      | 	vis{7}='off';
      | else								%output of HandInTarget block is an array
      | 	vis{4}='on';
      | 	vis{5}='on';
      | 	vis{6}='on';
      | 	vis{7}='on';
      | end
      | set_param(block_path,'MaskVisibilities',vis);
      mask TypeOptions source: dialog | port
      mask Callback source:
      | % Show or hide the opacity input on the mask dialog
      | sourceStr=get_param(gcb,'source');
      | vis=get_param(gcb,'MaskVisibilities');
      | 
      | if strmatch(sourceStr, 'dialog')
      | 	vis{10}='on';
      | else
      | 	vis{10}='off';
      | end
      | 
      | set_param(gcb,'MaskVisibilities',vis);
      mask TypeOptions target_display: Both subject and operator displays | Subject display only | Operator display only
      mask Display: disp(columntext); port_label('output',1,outputname); port_label('input',1, inputname1); port_label('input',2, inputname2);
  Draw_Start : Subsystem  AncestorBlock=Video/Show_Target_With_Label  mask(Show_Target_With_Label){target_type=Circle, num_states=1, attribcol1=[TARGET_COLOR TARGET_COLOR TARGET_STROKE TARGET_RADIUS 0 0 0], attribcol2=[6 6 0 3 0 0 0], attribcol3=[0 0 0 0 0 0 0], attribcol4=[0 0 0 0 0 0 0], attribcol5=[0 0 24 0 0 0 0], stateindices_padding=[0 0 0 0;0 0 0 0;0 0 0 0;0 0 0 0;0 0 0 0], source=dialog, opacity=100, target_display=Both subject and operator displays}
      mask prompts: target_type "Type of Target"; num_states "Number of Target States"; attribcol1 "State 1 Target Table Column(s)"; attribcol2 "State 2 Target Table Column(s)"; attribcol3 "State 3 Target Table Column(s)"; attribcol4 "State 4 Target Table Column(s)"; attribcol5 "State 5 Target Table Column(s)"; stateindices_padding "State Indices Padding"; source "Source for Opacity"; target_display "Target Display"
      mask help: This block returns a VCODE that, when sent to the Process_Video_CMD block, will cause a single target with a text label to be drawn. The label will be centered at the centroid of the target. Target parameters are specified in the Target Table according to the columns defined below and the row input to this block.
      mask init: same as BimanualCarvingModifiedOldEMG/Draw_Hand_Endpoint
      mask Help:
      | Used to draw a single, stationary target with a label.
      | 
      | <H2>Library </H2>
      | Video
      | 
      | <H2>Description </H2>
      | This block returns a VCODE, which when sent to the Process_Video_CMD block will draw a single stationary target with a label. The VCODE contains all of the target parameters necessary to draw the target and the label.
      | <P>
      | The VCODE is generated from information contained in the Target Table. Which parts of the Target Table are used is determined by the columns selected (see Parameters and Dialog Box below).<P>
      | 
      | <p>For example, assume the "row" input is 2, the "type of target" is set to "rectangle" and the "Target Table Columns" is set to [3 0 0 4 5 0 6 7 4].
      | Then using the sample target table below a red rectangle will be drawn at (20cm, 40cm) with a width of 10cm and a height of 3cm.
      | The rectangle will have the word "Maybe" in yellow on it in letters 3cm heigh. The zeros in the  "Target Table Columns" indicate those parameters are not used (i.e. no stroke color, no stroke width, and no rotation).
      | 
      | <p><tt>
      | ______________________________________________________________________<br>
      | |&nbsp;&nbsp;&nbsp;&nbsp;&nbsp;&nbsp;&nbsp;&nbsp;&nbsp;&nbsp;| X Pos | Y pos |&nbsp;&nbsp;Fill | Width | Height |&nbsp;&nbsp;Text | TColor |<br>
      | ----------------------------------------------------------------------<br>
      | | target 1 |&nbsp;&nbsp;&nbsp;&nbsp;10 |&nbsp;&nbsp;&nbsp;&nbsp;10 | white |&nbsp;&nbsp;&nbsp;&nbsp;&nbsp;5 |&nbsp;&nbsp;&nbsp;&nbsp;&nbsp;&nbsp;2 |&nbsp;&nbsp;&nbsp;Yes |&nbsp;&nbsp;green |<br>
      | | target 2 |&nbsp;&nbsp;&nbsp;&nbsp;20 |&nbsp;&nbsp;&nbsp;&nbsp;40 |&nbsp;&nbsp;&nbsp;red |&nbsp;&nbsp;&nbsp;&nbsp;10 |&nbsp;&nbsp;&nbsp;&nbsp;&nbsp;&nbsp;3 | Maybe | yellow |<br>
      | | target 3 |&nbsp;&nbsp;&nbsp;-40 |&nbsp;&nbsp;&nbsp;&nbsp;10 |&nbsp;&nbsp;blue |&nbsp;&nbsp;&nbsp;&nbsp;&nbsp;3 |&nbsp;&nbsp;&nbsp;&nbsp;&nbsp;&nbsp;4 | Wrong |&nbsp;&nbsp;&nbsp;&nbsp;red |
      | ----------------------------------------------------------------------<br>
      | 
      | 
      | </tt>
      | 
      | 
      | <p>Inputs:<br>
      | <B> Target_Row: </B> this scalar input determines which row in the Target Table is used to define the target parameters. Typically the Target_Row comes from the Trial_Protocol.  <P>
      | <B> Target_State: </B> this scalar input determines which state the target is in. Different states reference different columns in the Target Table (as defined in the Dialog Box). Typically the Target_State input is controlled by the Stateflow chart to dynamically change the appearance of the target depending on system and/or subject behavior. Target_State=0 is a valid input, which turns the target off. The intended method for turning a target off is to set Target_State=0. <BR>
      | <P>
      | <B>Opacity:</B> This input is only available if Source for Opacity is selected as port, in which case the opacity for all of the targets created by this block is specified as a percentage.
      | The length of this input must either match the length of the Target_Row(s) input (i.e. which case each Opacity maps to the appropriate Target_row)
      | or this input must be a scalar (in which case the Opacity maps to all of the Target_Rows).<BR>
      | <P>
      | There is one output from this block:
      | <P>
      | <B> VCODE: </B> this output is a vector containing one VCODE. This output must go to the Process_Video_CMD block of the video library for the target to actually be shown (if any other visual targets are to be displayed, then this VCODE output must be concatenated with the other VCODES prior to connection to the Process_Video_CMD block - see Help for the Process_Video_CMD block for more information).
      | <P>
      | To show multiple targets simultaneously, multiple copies of the Show_Target and Show_Target_With_Label blocks can be used in a Task Program. The output VCODES from multiple Show_Target and Show_Target_With_Label blocks must be concatenated prior to connection to the Process_Video_CMD block.
      | <P>
      | 
      | <H2>Parameters and Dialog Box</H2>
      | <B>Type of Target:</B> Choose the type of target specified in the target table.
      | <P>
      | <B>Number of Target States:</B> Choose the number of target states specified in each target row. Up to five target states are allowed per target row.
      | <P>
      | <B>State [n] Target Table Columns:</B> Enter the column indices that specify the relevant target attributes in the Target Table. All target types have the same first three target attributes (fill colour, stroke colour and stroke width) and the same last three target attributes (label text, label colour, and label height).
      | <Blockquote>
      | <P>
      | Element 1 (fill colour) - points to the column index in the Target Table containing the fill colour. If this index is 0, then the fill colour is transparent and the Target Table is not referenced. For line targets, the fill colour is not used.
      | <P>
      | Element 2 (stroke colour) - points to the column index in the Target Table containing the stroke colour. If this index is 0, then the stroke colour is transparent and the Target Table is not referenced. It is possible to use the same column index for both fill colour and stroke colour (i.e.  if single-colour targets are desired). For line targets, stroke colour defines the colour of the line.
      | <P>
      | Element 3 (stroke width) - points to the column index in the Target Table containing the stroke width (cm). If no stroke is desired, then setting the stroke column index to 0 will produce a stroke width of 0  and the Target Table is not referenced.  Setting stroke column index to a value less than 0 will produce a standard 1 mm stroke width, again without referencing the Target Table. For line targets, stroke width defines the width of the line.
      | <P>
      | <B><I>Circle</I></B> <P>
      | Element 4 (radius) - radius of the circle (cm).
      | <P>
      | <B><I>Ellipse</I></B> <P>
      | Elements 4-6 (ellipse properties) - major radius (cm), minor radius (cm), rotation angle (degrees). If no rotation is desired, then setting rotation column index to 0 will produce a default rotation of 0 and the Target Table will not be referenced.
      | <P>
      | <B><I>Rectangle</I></B><P>
      | Elements 4-6 (rectangle properties) - length (cm), height (cm), rotation angle (degrees). If no rotation is desired, then setting rotation column index to 0 will produce a default rotation of 0 and the Target Table will not be referenced.
      | <P>
      | <B><I>Line</I></B><P>
      | Elements 4-5 (line properties) - end point x-axis position relative to start point (cm), end point y-axis position relative to start point (cm). The width and colour of the line are defined by the stroke width and the stroke colour, respectively. The fill colour column is ignored (i.e. any value can be used for column 1)
      | <P>
      | <B><I>Triangle</I></B><P>
      | Elements 4-7 (triangle properties) - length (cm), height (cm), offset of peak of triangle relative to midpoint of the length (cm), rotation angle (degrees). If a height column index of 0 is specified, then an equilateral triangle with sides of the specified length will be created and the Target Table will not be referenced for height or peak offset. If no rotation is desired, then setting a rotation column index of 0 will produce a default rotation of 0 and the Target Table will not be referenced.
      | <P>
      | <B><I>Label</I></B>
      | <P>
      | The last three elements of the target state vector define the label. In order, these elements are:
      | <P>
      | Label text - the index of the column in the Target Table containing the text used for the label (up to 50 characters).
      | <P>
      | Label colour - the index of the column in the Target Table containing the label colour. If this index is 0, then the label colour is transparent and the Target Table is not referenced.
      | <P>
      | Label height - the index of the column in the Target Table containing the label height (cm).
      | </Blockquote>
      | <P>
      | Each target state requires its own set of column index definitions (although multiple states can point to the same column index if desired).<P>
      | 
      | <B>Source for Opacity:</B> Choose either dialog, to specify the opacity in this dialog, or port, which will create a new input to allow dynamic control of opacity.
      | <P>
      | <B>Opacity:</B> This parameter is only available if Source for Opacity is selected as dialog, in which case the opacity for all of the targets created by this block is specified as a percentage.
      | <P>
      | <B>Target Display:</B> This option determines whether the target(s) are shown on the operator display only, the subject display only, or both displays.
      | <P>
      | 
      | <H2>Examples</H2>
      | 
      | <B>Example 1:</B>  Suppose a target row will be used to define 1 state for an ellipse type target. It will be an outline of an ellipse with a label in the center (using a stroke colour and a standard 1mm stroke width). The related Target Table columns are:
      | <P>
      | column 4 = colour<BR>
      | column 5 = major radius<BR>
      | column 6 = minor radius<BR>
      | column 7 = orientation<BR>
      | column 8 = label text<BR>
      | column 9 = label colour<BR>
      | column 10 = label height
      | <P>For this example, "State 1 Target Table Columns" would equal [0 4 -1 5 6 7 8 9 10].
      | <P>
      | 
      | <H2>Related Blocks </H2>
      | Show_Target<BR>
      | Process_Video_CMD
      mask TypeOptions target_type: Circle | Ellipse | Rectangle | Line | Triangle
      mask Callback target_type:
      | %%%%
      | % Because of bugs iN R2007, R2010a and R2013a (which have been reported to Mathworks), the following code
      | % is required here because in the Initialization Section it will ONLY correctly update those Mask Parameters that are hidden
      | % when the OK button is clicked (NOTE: the initialization code will correctly update all Mask Parameters when the Apply button
      | % is clicked, the bug is that it should also update everything when the OK button is clicked in the absence of an Apply click)
      | %
      | % Adding a set_param call which updates one of the mask parameters will call the initialization code to run, which "avoids"
      | % this bug. This code should be removed once Mathworks has fixed this bug.
      | 
      | temp = get_param(gcb, 'target_type');
      | set_param(gcb, 'target_type', temp);
      mask TypeOptions num_states: 1 | 2 | 3 | 4 | 5
      mask Callback num_states:
      | block_path=gcb;
      | num_states=str2num(get_param(block_path, 'num_states'));
      | vis=get_param(block_path,'MaskVisibilities');
      | 
      | %If the number of states>1, then output an array instead of a vector.
      | %Only show those inputs necessary on the Mask
      | output_block=char(find_system(block_path,'LookUnderMasks','all','SearchDepth',1,'BlockType','Outport'));
      | if num_states==1			%output of HandInTarget block is a vector
      | 	vis{4}='off';
      | 	vis{5}='off';
      | 	vis{6}='off';
      | 	vis{7}='off';
      | elseif num_states==2					%output of HandInTarget block is an array
      | 	vis{4}='on';
      | 	vis{5}='off';
      | 	vis{6}='off';
      | 	vis{7}='off';
      | elseif num_states==3					%output of HandInTarget block is an array
      | 	vis{4}='on';
      | 	vis{5}='on';
      | 	vis{6}='off';
      | 	vis{7}='off';
      | elseif num_states==4					%output of HandInTarget block is an array
      | 	vis{4}='on';
      | 	vis{5}='on';
      | 	vis{6}='on';
      | 	vis{7}='off';
      | else								%output of HandInTarget block is an array
      | 	vis{4}='on';
      | 	vis{5}='on';
      | 	vis{6}='on';
      | 	vis{7}='on';
      | end
      | set_param(block_path,'MaskVisibilities',vis);
      mask TypeOptions source: dialog | port
      mask Callback source:
      | % Show or hide the opacity input on the mask dialog
      | sourceStr=get_param(gcb,'source');
      | vis=get_param(gcb,'MaskVisibilities');
      | 
      | if strmatch(sourceStr, 'dialog')
      | 	vis{10}='on';
      | else
      | 	vis{10}='off';
      | end
      | 
      | set_param(gcb,'MaskVisibilities',vis);
      mask TypeOptions target_display: Both subject and operator displays | Subject display only | Operator display only
      mask Display: disp(columntext); port_label('output',1,outputname); port_label('input',1, inputname1); port_label('input',2, inputname2);
  Draw_finish_line : Subsystem  AncestorBlock=Video/Show_Target_With_Label  mask(Show_Target_With_Label){target_type=Line, num_states=1, attribcol1=[HAND_COLOR HAND_COLOR TARGET_STROKE TARGET_RADIUS 0 0 0 0], attribcol2=[6 6 0 3 0 0 0 0], attribcol3=[0 0 0 0 0 0 0 0], attribcol4=[0 0 0 0 0 0 0 0], attribcol5=[0 0 24 0 0 0 0 0], stateindices_padding=[0 0 0;0 0 0;0 0 0;0 0 0;0 0 0], source=dialog, opacity=100, target_display=Both subject and operator displays}
      mask prompts: target_type "Type of Target"; num_states "Number of Target States"; attribcol1 "State 1 Target Table Column(s)"; attribcol2 "State 2 Target Table Column(s)"; attribcol3 "State 3 Target Table Column(s)"; attribcol4 "State 4 Target Table Column(s)"; attribcol5 "State 5 Target Table Column(s)"; stateindices_padding "State Indices Padding"; source "Source for Opacity"; target_display "Target Display"
      mask help: This block returns a VCODE that, when sent to the Process_Video_CMD block, will cause a single target with a text label to be drawn. The label will be centered at the centroid of the target. Target parameters are specified in the Target Table according to the columns defined below and the row input to this block.
      mask init: same as BimanualCarvingModifiedOldEMG/Draw_Hand_Endpoint
      mask Help:
      | Used to draw a single, stationary target with a label.
      | 
      | <H2>Library </H2>
      | Video
      | 
      | <H2>Description </H2>
      | This block returns a VCODE, which when sent to the Process_Video_CMD block will draw a single stationary target with a label. The VCODE contains all of the target parameters necessary to draw the target and the label.
      | <P>
      | The VCODE is generated from information contained in the Target Table. Which parts of the Target Table are used is determined by the columns selected (see Parameters and Dialog Box below).<P>
      | 
      | <p>For example, assume the "row" input is 2, the "type of target" is set to "rectangle" and the "Target Table Columns" is set to [3 0 0 4 5 0 6 7 4].
      | Then using the sample target table below a red rectangle will be drawn at (20cm, 40cm) with a width of 10cm and a height of 3cm.
      | The rectangle will have the word "Maybe" in yellow on it in letters 3cm heigh. The zeros in the  "Target Table Columns" indicate those parameters are not used (i.e. no stroke color, no stroke width, and no rotation).
      | 
      | <p><tt>
      | ______________________________________________________________________<br>
      | |&nbsp;&nbsp;&nbsp;&nbsp;&nbsp;&nbsp;&nbsp;&nbsp;&nbsp;&nbsp;| X Pos | Y pos |&nbsp;&nbsp;Fill | Width | Height |&nbsp;&nbsp;Text | TColor |<br>
      | ----------------------------------------------------------------------<br>
      | | target 1 |&nbsp;&nbsp;&nbsp;&nbsp;10 |&nbsp;&nbsp;&nbsp;&nbsp;10 | white |&nbsp;&nbsp;&nbsp;&nbsp;&nbsp;5 |&nbsp;&nbsp;&nbsp;&nbsp;&nbsp;&nbsp;2 |&nbsp;&nbsp;&nbsp;Yes |&nbsp;&nbsp;green |<br>
      | | target 2 |&nbsp;&nbsp;&nbsp;&nbsp;20 |&nbsp;&nbsp;&nbsp;&nbsp;40 |&nbsp;&nbsp;&nbsp;red |&nbsp;&nbsp;&nbsp;&nbsp;10 |&nbsp;&nbsp;&nbsp;&nbsp;&nbsp;&nbsp;3 | Maybe | yellow |<br>
      | | target 3 |&nbsp;&nbsp;&nbsp;-40 |&nbsp;&nbsp;&nbsp;&nbsp;10 |&nbsp;&nbsp;blue |&nbsp;&nbsp;&nbsp;&nbsp;&nbsp;3 |&nbsp;&nbsp;&nbsp;&nbsp;&nbsp;&nbsp;4 | Wrong |&nbsp;&nbsp;&nbsp;&nbsp;red |
      | ----------------------------------------------------------------------<br>
      | 
      | 
      | </tt>
      | 
      | 
      | <p>Inputs:<br>
      | <B> Target_Row: </B> this scalar input determines which row in the Target Table is used to define the target parameters. Typically the Target_Row comes from the Trial_Protocol.  <P>
      | <B> Target_State: </B> this scalar input determines which state the target is in. Different states reference different columns in the Target Table (as defined in the Dialog Box). Typically the Target_State input is controlled by the Stateflow chart to dynamically change the appearance of the target depending on system and/or subject behavior. Target_State=0 is a valid input, which turns the target off. The intended method for turning a target off is to set Target_State=0. <BR>
      | <P>
      | <B>Opacity:</B> This input is only available if Source for Opacity is selected as port, in which case the opacity for all of the targets created by this block is specified as a percentage.
      | The length of this input must either match the length of the Target_Row(s) input (i.e. which case each Opacity maps to the appropriate Target_row)
      | or this input must be a scalar (in which case the Opacity maps to all of the Target_Rows).<BR>
      | <P>
      | There is one output from this block:
      | <P>
      | <B> VCODE: </B> this output is a vector containing one VCODE. This output must go to the Process_Video_CMD block of the video library for the target to actually be shown (if any other visual targets are to be displayed, then this VCODE output must be concatenated with the other VCODES prior to connection to the Process_Video_CMD block - see Help for the Process_Video_CMD block for more information).
      | <P>
      | To show multiple targets simultaneously, multiple copies of the Show_Target and Show_Target_With_Label blocks can be used in a Task Program. The output VCODES from multiple Show_Target and Show_Target_With_Label blocks must be concatenated prior to connection to the Process_Video_CMD block.
      | <P>
      | 
      | <H2>Parameters and Dialog Box</H2>
      | <B>Type of Target:</B> Choose the type of target specified in the target table.
      | <P>
      | <B>Number of Target States:</B> Choose the number of target states specified in each target row. Up to five target states are allowed per target row.
      | <P>
      | <B>State [n] Target Table Columns:</B> Enter the column indices that specify the relevant target attributes in the Target Table. All target types have the same first three target attributes (fill colour, stroke colour and stroke width) and the same last three target attributes (label text, label colour, and label height).
      | <Blockquote>
      | <P>
      | Element 1 (fill colour) - points to the column index in the Target Table containing the fill colour. If this index is 0, then the fill colour is transparent and the Target Table is not referenced. For line targets, the fill colour is not used.
      | <P>
      | Element 2 (stroke colour) - points to the column index in the Target Table containing the stroke colour. If this index is 0, then the stroke colour is transparent and the Target Table is not referenced. It is possible to use the same column index for both fill colour and stroke colour (i.e.  if single-colour targets are desired). For line targets, stroke colour defines the colour of the line.
      | <P>
      | Element 3 (stroke width) - points to the column index in the Target Table containing the stroke width (cm). If no stroke is desired, then setting the stroke column index to 0 will produce a stroke width of 0  and the Target Table is not referenced.  Setting stroke column index to a value less than 0 will produce a standard 1 mm stroke width, again without referencing the Target Table. For line targets, stroke width defines the width of the line.
      | <P>
      | <B><I>Circle</I></B> <P>
      | Element 4 (radius) - radius of the circle (cm).
      | <P>
      | <B><I>Ellipse</I></B> <P>
      | Elements 4-6 (ellipse properties) - major radius (cm), minor radius (cm), rotation angle (degrees). If no rotation is desired, then setting rotation column index to 0 will produce a default rotation of 0 and the Target Table will not be referenced.
      | <P>
      | <B><I>Rectangle</I></B><P>
      | Elements 4-6 (rectangle properties) - length (cm), height (cm), rotation angle (degrees). If no rotation is desired, then setting rotation column index to 0 will produce a default rotation of 0 and the Target Table will not be referenced.
      | <P>
      | <B><I>Line</I></B><P>
      | Elements 4-5 (line properties) - end point x-axis position relative to start point (cm), end point y-axis position relative to start point (cm). The width and colour of the line are defined by the stroke width and the stroke colour, respectively. The fill colour column is ignored (i.e. any value can be used for column 1)
      | <P>
      | <B><I>Triangle</I></B><P>
      | Elements 4-7 (triangle properties) - length (cm), height (cm), offset of peak of triangle relative to midpoint of the length (cm), rotation angle (degrees). If a height column index of 0 is specified, then an equilateral triangle with sides of the specified length will be created and the Target Table will not be referenced for height or peak offset. If no rotation is desired, then setting a rotation column index of 0 will produce a default rotation of 0 and the Target Table will not be referenced.
      | <P>
      | <B><I>Label</I></B>
      | <P>
      | The last three elements of the target state vector define the label. In order, these elements are:
      | <P>
      | Label text - the index of the column in the Target Table containing the text used for the label (up to 50 characters).
      | <P>
      | Label colour - the index of the column in the Target Table containing the label colour. If this index is 0, then the label colour is transparent and the Target Table is not referenced.
      | <P>
      | Label height - the index of the column in the Target Table containing the label height (cm).
      | </Blockquote>
      | <P>
      | Each target state requires its own set of column index definitions (although multiple states can point to the same column index if desired).<P>
      | 
      | <B>Source for Opacity:</B> Choose either dialog, to specify the opacity in this dialog, or port, which will create a new input to allow dynamic control of opacity.
      | <P>
      | <B>Opacity:</B> This parameter is only available if Source for Opacity is selected as dialog, in which case the opacity for all of the targets created by this block is specified as a percentage.
      | <P>
      | <B>Target Display:</B> This option determines whether the target(s) are shown on the operator display only, the subject display only, or both displays.
      | <P>
      | 
      | <H2>Examples</H2>
      | 
      | <B>Example 1:</B>  Suppose a target row will be used to define 1 state for an ellipse type target. It will be an outline of an ellipse with a label in the center (using a stroke colour and a standard 1mm stroke width). The related Target Table columns are:
      | <P>
      | column 4 = colour<BR>
      | column 5 = major radius<BR>
      | column 6 = minor radius<BR>
      | column 7 = orientation<BR>
      | column 8 = label text<BR>
      | column 9 = label colour<BR>
      | column 10 = label height
      | <P>For this example, "State 1 Target Table Columns" would equal [0 4 -1 5 6 7 8 9 10].
      | <P>
      | 
      | <H2>Related Blocks </H2>
      | Show_Target<BR>
      | Process_Video_CMD
      mask TypeOptions target_type: Circle | Ellipse | Rectangle | Line | Triangle
      mask Callback target_type:
      | %%%%
      | % Because of bugs iN R2007, R2010a and R2013a (which have been reported to Mathworks), the following code
      | % is required here because in the Initialization Section it will ONLY correctly update those Mask Parameters that are hidden
      | % when the OK button is clicked (NOTE: the initialization code will correctly update all Mask Parameters when the Apply button
      | % is clicked, the bug is that it should also update everything when the OK button is clicked in the absence of an Apply click)
      | %
      | % Adding a set_param call which updates one of the mask parameters will call the initialization code to run, which "avoids"
      | % this bug. This code should be removed once Mathworks has fixed this bug.
      | 
      | temp = get_param(gcb, 'target_type');
      | set_param(gcb, 'target_type', temp);
      mask TypeOptions num_states: 1 | 2 | 3 | 4 | 5
      mask Callback num_states:
      | block_path=gcb;
      | num_states=str2num(get_param(block_path, 'num_states'));
      | vis=get_param(block_path,'MaskVisibilities');
      | 
      | %If the number of states>1, then output an array instead of a vector.
      | %Only show those inputs necessary on the Mask
      | output_block=char(find_system(block_path,'LookUnderMasks','all','SearchDepth',1,'BlockType','Outport'));
      | if num_states==1			%output of HandInTarget block is a vector
      | 	vis{4}='off';
      | 	vis{5}='off';
      | 	vis{6}='off';
      | 	vis{7}='off';
      | elseif num_states==2					%output of HandInTarget block is an array
      | 	vis{4}='on';
      | 	vis{5}='off';
      | 	vis{6}='off';
      | 	vis{7}='off';
      | elseif num_states==3					%output of HandInTarget block is an array
      | 	vis{4}='on';
      | 	vis{5}='on';
      | 	vis{6}='off';
      | 	vis{7}='off';
      | elseif num_states==4					%output of HandInTarget block is an array
      | 	vis{4}='on';
      | 	vis{5}='on';
      | 	vis{6}='on';
      | 	vis{7}='off';
      | else								%output of HandInTarget block is an array
      | 	vis{4}='on';
      | 	vis{5}='on';
      | 	vis{6}='on';
      | 	vis{7}='on';
      | end
      | set_param(block_path,'MaskVisibilities',vis);
      mask TypeOptions source: dialog | port
      mask Callback source:
      | % Show or hide the opacity input on the mask dialog
      | sourceStr=get_param(gcb,'source');
      | vis=get_param(gcb,'MaskVisibilities');
      | 
      | if strmatch(sourceStr, 'dialog')
      | 	vis{10}='on';
      | else
      | 	vis{10}='off';
      | end
      | 
      | set_param(gcb,'MaskVisibilities',vis);
      mask TypeOptions target_display: Both subject and operator displays | Subject display only | Operator display only
      mask Display: disp(columntext); port_label('output',1,outputname); port_label('input',1, inputname1); port_label('input',2, inputname2);
  Draw_message : Subsystem  AncestorBlock=Video/Show_Target_With_Label  mask(Show_Target_With_Label){target_type=Rectangle, num_states=1, attribcol1=[HAND_COLOR HAND_COLOR 0 HAND_RADIUS HAND_RADIUS 0 0 0 0], attribcol2=[6 6 0 3 0 0 0 0 0], attribcol3=[0 0 0 0 0 0 0 0 0], attribcol4=[0 0 0 0 0 0 0 0 0], attribcol5=[0 0 24 0 0 0 0 0 0], stateindices_padding=[0 0;0 0;0 0;0 0;0 0], source=dialog, opacity=100, target_display=Both subject and operator displays}
      mask prompts: target_type "Type of Target"; num_states "Number of Target States"; attribcol1 "State 1 Target Table Column(s)"; attribcol2 "State 2 Target Table Column(s)"; attribcol3 "State 3 Target Table Column(s)"; attribcol4 "State 4 Target Table Column(s)"; attribcol5 "State 5 Target Table Column(s)"; stateindices_padding "State Indices Padding"; source "Source for Opacity"; target_display "Target Display"
      mask help: This block returns a VCODE that, when sent to the Process_Video_CMD block, will cause a single target with a text label to be drawn. The label will be centered at the centroid of the target. Target parameters are specified in the Target Table according to the columns defined below and the row input to this block.
      mask init: same as BimanualCarvingModifiedOldEMG/Draw_Hand_Endpoint
      mask Help:
      | Used to draw a single, stationary target with a label.
      | 
      | <H2>Library </H2>
      | Video
      | 
      | <H2>Description </H2>
      | This block returns a VCODE, which when sent to the Process_Video_CMD block will draw a single stationary target with a label. The VCODE contains all of the target parameters necessary to draw the target and the label.
      | <P>
      | The VCODE is generated from information contained in the Target Table. Which parts of the Target Table are used is determined by the columns selected (see Parameters and Dialog Box below).<P>
      | 
      | <p>For example, assume the "row" input is 2, the "type of target" is set to "rectangle" and the "Target Table Columns" is set to [3 0 0 4 5 0 6 7 4].
      | Then using the sample target table below a red rectangle will be drawn at (20cm, 40cm) with a width of 10cm and a height of 3cm.
      | The rectangle will have the word "Maybe" in yellow on it in letters 3cm heigh. The zeros in the  "Target Table Columns" indicate those parameters are not used (i.e. no stroke color, no stroke width, and no rotation).
      | 
      | <p><tt>
      | ______________________________________________________________________<br>
      | |&nbsp;&nbsp;&nbsp;&nbsp;&nbsp;&nbsp;&nbsp;&nbsp;&nbsp;&nbsp;| X Pos | Y pos |&nbsp;&nbsp;Fill | Width | Height |&nbsp;&nbsp;Text | TColor |<br>
      | ----------------------------------------------------------------------<br>
      | | target 1 |&nbsp;&nbsp;&nbsp;&nbsp;10 |&nbsp;&nbsp;&nbsp;&nbsp;10 | white |&nbsp;&nbsp;&nbsp;&nbsp;&nbsp;5 |&nbsp;&nbsp;&nbsp;&nbsp;&nbsp;&nbsp;2 |&nbsp;&nbsp;&nbsp;Yes |&nbsp;&nbsp;green |<br>
      | | target 2 |&nbsp;&nbsp;&nbsp;&nbsp;20 |&nbsp;&nbsp;&nbsp;&nbsp;40 |&nbsp;&nbsp;&nbsp;red |&nbsp;&nbsp;&nbsp;&nbsp;10 |&nbsp;&nbsp;&nbsp;&nbsp;&nbsp;&nbsp;3 | Maybe | yellow |<br>
      | | target 3 |&nbsp;&nbsp;&nbsp;-40 |&nbsp;&nbsp;&nbsp;&nbsp;10 |&nbsp;&nbsp;blue |&nbsp;&nbsp;&nbsp;&nbsp;&nbsp;3 |&nbsp;&nbsp;&nbsp;&nbsp;&nbsp;&nbsp;4 | Wrong |&nbsp;&nbsp;&nbsp;&nbsp;red |
      | ----------------------------------------------------------------------<br>
      | 
      | 
      | </tt>
      | 
      | 
      | <p>Inputs:<br>
      | <B> Target_Row: </B> this scalar input determines which row in the Target Table is used to define the target parameters. Typically the Target_Row comes from the Trial_Protocol.  <P>
      | <B> Target_State: </B> this scalar input determines which state the target is in. Different states reference different columns in the Target Table (as defined in the Dialog Box). Typically the Target_State input is controlled by the Stateflow chart to dynamically change the appearance of the target depending on system and/or subject behavior. Target_State=0 is a valid input, which turns the target off. The intended method for turning a target off is to set Target_State=0. <BR>
      | <P>
      | <B>Opacity:</B> This input is only available if Source for Opacity is selected as port, in which case the opacity for all of the targets created by this block is specified as a percentage.
      | The length of this input must either match the length of the Target_Row(s) input (i.e. which case each Opacity maps to the appropriate Target_row)
      | or this input must be a scalar (in which case the Opacity maps to all of the Target_Rows).<BR>
      | <P>
      | There is one output from this block:
      | <P>
      | <B> VCODE: </B> this output is a vector containing one VCODE. This output must go to the Process_Video_CMD block of the video library for the target to actually be shown (if any other visual targets are to be displayed, then this VCODE output must be concatenated with the other VCODES prior to connection to the Process_Video_CMD block - see Help for the Process_Video_CMD block for more information).
      | <P>
      | To show multiple targets simultaneously, multiple copies of the Show_Target and Show_Target_With_Label blocks can be used in a Task Program. The output VCODES from multiple Show_Target and Show_Target_With_Label blocks must be concatenated prior to connection to the Process_Video_CMD block.
      | <P>
      | 
      | <H2>Parameters and Dialog Box</H2>
      | <B>Type of Target:</B> Choose the type of target specified in the target table.
      | <P>
      | <B>Number of Target States:</B> Choose the number of target states specified in each target row. Up to five target states are allowed per target row.
      | <P>
      | <B>State [n] Target Table Columns:</B> Enter the column indices that specify the relevant target attributes in the Target Table. All target types have the same first three target attributes (fill colour, stroke colour and stroke width) and the same last three target attributes (label text, label colour, and label height).
      | <Blockquote>
      | <P>
      | Element 1 (fill colour) - points to the column index in the Target Table containing the fill colour. If this index is 0, then the fill colour is transparent and the Target Table is not referenced. For line targets, the fill colour is not used.
      | <P>
      | Element 2 (stroke colour) - points to the column index in the Target Table containing the stroke colour. If this index is 0, then the stroke colour is transparent and the Target Table is not referenced. It is possible to use the same column index for both fill colour and stroke colour (i.e.  if single-colour targets are desired). For line targets, stroke colour defines the colour of the line.
      | <P>
      | Element 3 (stroke width) - points to the column index in the Target Table containing the stroke width (cm). If no stroke is desired, then setting the stroke column index to 0 will produce a stroke width of 0  and the Target Table is not referenced.  Setting stroke column index to a value less than 0 will produce a standard 1 mm stroke width, again without referencing the Target Table. For line targets, stroke width defines the width of the line.
      | <P>
      | <B><I>Circle</I></B> <P>
      | Element 4 (radius) - radius of the circle (cm).
      | <P>
      | <B><I>Ellipse</I></B> <P>
      | Elements 4-6 (ellipse properties) - major radius (cm), minor radius (cm), rotation angle (degrees). If no rotation is desired, then setting rotation column index to 0 will produce a default rotation of 0 and the Target Table will not be referenced.
      | <P>
      | <B><I>Rectangle</I></B><P>
      | Elements 4-6 (rectangle properties) - length (cm), height (cm), rotation angle (degrees). If no rotation is desired, then setting rotation column index to 0 will produce a default rotation of 0 and the Target Table will not be referenced.
      | <P>
      | <B><I>Line</I></B><P>
      | Elements 4-5 (line properties) - end point x-axis position relative to start point (cm), end point y-axis position relative to start point (cm). The width and colour of the line are defined by the stroke width and the stroke colour, respectively. The fill colour column is ignored (i.e. any value can be used for column 1)
      | <P>
      | <B><I>Triangle</I></B><P>
      | Elements 4-7 (triangle properties) - length (cm), height (cm), offset of peak of triangle relative to midpoint of the length (cm), rotation angle (degrees). If a height column index of 0 is specified, then an equilateral triangle with sides of the specified length will be created and the Target Table will not be referenced for height or peak offset. If no rotation is desired, then setting a rotation column index of 0 will produce a default rotation of 0 and the Target Table will not be referenced.
      | <P>
      | <B><I>Label</I></B>
      | <P>
      | The last three elements of the target state vector define the label. In order, these elements are:
      | <P>
      | Label text - the index of the column in the Target Table containing the text used for the label (up to 50 characters).
      | <P>
      | Label colour - the index of the column in the Target Table containing the label colour. If this index is 0, then the label colour is transparent and the Target Table is not referenced.
      | <P>
      | Label height - the index of the column in the Target Table containing the label height (cm).
      | </Blockquote>
      | <P>
      | Each target state requires its own set of column index definitions (although multiple states can point to the same column index if desired).<P>
      | 
      | <B>Source for Opacity:</B> Choose either dialog, to specify the opacity in this dialog, or port, which will create a new input to allow dynamic control of opacity.
      | <P>
      | <B>Opacity:</B> This parameter is only available if Source for Opacity is selected as dialog, in which case the opacity for all of the targets created by this block is specified as a percentage.
      | <P>
      | <B>Target Display:</B> This option determines whether the target(s) are shown on the operator display only, the subject display only, or both displays.
      | <P>
      | 
      | <H2>Examples</H2>
      | 
      | <B>Example 1:</B>  Suppose a target row will be used to define 1 state for an ellipse type target. It will be an outline of an ellipse with a label in the center (using a stroke colour and a standard 1mm stroke width). The related Target Table columns are:
      | <P>
      | column 4 = colour<BR>
      | column 5 = major radius<BR>
      | column 6 = minor radius<BR>
      | column 7 = orientation<BR>
      | column 8 = label text<BR>
      | column 9 = label colour<BR>
      | column 10 = label height
      | <P>For this example, "State 1 Target Table Columns" would equal [0 4 -1 5 6 7 8 9 10].
      | <P>
      | 
      | <H2>Related Blocks </H2>
      | Show_Target<BR>
      | Process_Video_CMD
      mask TypeOptions target_type: Circle | Ellipse | Rectangle | Line | Triangle
      mask Callback target_type:
      | %%%%
      | % Because of bugs iN R2007, R2010a and R2013a (which have been reported to Mathworks), the following code
      | % is required here because in the Initialization Section it will ONLY correctly update those Mask Parameters that are hidden
      | % when the OK button is clicked (NOTE: the initialization code will correctly update all Mask Parameters when the Apply button
      | % is clicked, the bug is that it should also update everything when the OK button is clicked in the absence of an Apply click)
      | %
      | % Adding a set_param call which updates one of the mask parameters will call the initialization code to run, which "avoids"
      | % this bug. This code should be removed once Mathworks has fixed this bug.
      | 
      | temp = get_param(gcb, 'target_type');
      | set_param(gcb, 'target_type', temp);
      mask TypeOptions num_states: 1 | 2 | 3 | 4 | 5
      mask Callback num_states:
      | block_path=gcb;
      | num_states=str2num(get_param(block_path, 'num_states'));
      | vis=get_param(block_path,'MaskVisibilities');
      | 
      | %If the number of states>1, then output an array instead of a vector.
      | %Only show those inputs necessary on the Mask
      | output_block=char(find_system(block_path,'LookUnderMasks','all','SearchDepth',1,'BlockType','Outport'));
      | if num_states==1			%output of HandInTarget block is a vector
      | 	vis{4}='off';
      | 	vis{5}='off';
      | 	vis{6}='off';
      | 	vis{7}='off';
      | elseif num_states==2					%output of HandInTarget block is an array
      | 	vis{4}='on';
      | 	vis{5}='off';
      | 	vis{6}='off';
      | 	vis{7}='off';
      | elseif num_states==3					%output of HandInTarget block is an array
      | 	vis{4}='on';
      | 	vis{5}='on';
      | 	vis{6}='off';
      | 	vis{7}='off';
      | elseif num_states==4					%output of HandInTarget block is an array
      | 	vis{4}='on';
      | 	vis{5}='on';
      | 	vis{6}='on';
      | 	vis{7}='off';
      | else								%output of HandInTarget block is an array
      | 	vis{4}='on';
      | 	vis{5}='on';
      | 	vis{6}='on';
      | 	vis{7}='on';
      | end
      | set_param(block_path,'MaskVisibilities',vis);
      mask TypeOptions source: dialog | port
      mask Callback source:
      | % Show or hide the opacity input on the mask dialog
      | sourceStr=get_param(gcb,'source');
      | vis=get_param(gcb,'MaskVisibilities');
      | 
      | if strmatch(sourceStr, 'dialog')
      | 	vis{10}='on';
      | else
      | 	vis{10}='off';
      | end
      | 
      | set_param(gcb,'MaskVisibilities',vis);
      mask TypeOptions target_display: Both subject and operator displays | Subject display only | Operator display only
      mask Display: disp(columntext); port_label('output',1,outputname); port_label('input',1, inputname1); port_label('input',2, inputname2);
  Draw_target : Subsystem  AncestorBlock=Video/Show_Target_With_Label  mask(Show_Target_With_Label){target_type=Line, num_states=1, attribcol1=[HAND_COLOR HAND_COLOR TARGET_STROKE TARGET_RADIUS 0 0 0 0], attribcol2=[6 6 0 3 0 0 0 0], attribcol3=[0 0 0 0 0 0 0 0], attribcol4=[0 0 0 0 0 0 0 0], attribcol5=[0 0 24 0 0 0 0 0], stateindices_padding=[0 0 0;0 0 0;0 0 0;0 0 0;0 0 0], source=dialog, opacity=100, target_display=Both subject and operator displays}
      mask prompts: target_type "Type of Target"; num_states "Number of Target States"; attribcol1 "State 1 Target Table Column(s)"; attribcol2 "State 2 Target Table Column(s)"; attribcol3 "State 3 Target Table Column(s)"; attribcol4 "State 4 Target Table Column(s)"; attribcol5 "State 5 Target Table Column(s)"; stateindices_padding "State Indices Padding"; source "Source for Opacity"; target_display "Target Display"
      mask help: This block returns a VCODE that, when sent to the Process_Video_CMD block, will cause a single target with a text label to be drawn. The label will be centered at the centroid of the target. Target parameters are specified in the Target Table according to the columns defined below and the row input to this block.
      mask init: same as BimanualCarvingModifiedOldEMG/Draw_Hand_Endpoint
      mask Help:
      | Used to draw a single, stationary target with a label.
      | 
      | <H2>Library </H2>
      | Video
      | 
      | <H2>Description </H2>
      | This block returns a VCODE, which when sent to the Process_Video_CMD block will draw a single stationary target with a label. The VCODE contains all of the target parameters necessary to draw the target and the label.
      | <P>
      | The VCODE is generated from information contained in the Target Table. Which parts of the Target Table are used is determined by the columns selected (see Parameters and Dialog Box below).<P>
      | 
      | <p>For example, assume the "row" input is 2, the "type of target" is set to "rectangle" and the "Target Table Columns" is set to [3 0 0 4 5 0 6 7 4].
      | Then using the sample target table below a red rectangle will be drawn at (20cm, 40cm) with a width of 10cm and a height of 3cm.
      | The rectangle will have the word "Maybe" in yellow on it in letters 3cm heigh. The zeros in the  "Target Table Columns" indicate those parameters are not used (i.e. no stroke color, no stroke width, and no rotation).
      | 
      | <p><tt>
      | ______________________________________________________________________<br>
      | |&nbsp;&nbsp;&nbsp;&nbsp;&nbsp;&nbsp;&nbsp;&nbsp;&nbsp;&nbsp;| X Pos | Y pos |&nbsp;&nbsp;Fill | Width | Height |&nbsp;&nbsp;Text | TColor |<br>
      | ----------------------------------------------------------------------<br>
      | | target 1 |&nbsp;&nbsp;&nbsp;&nbsp;10 |&nbsp;&nbsp;&nbsp;&nbsp;10 | white |&nbsp;&nbsp;&nbsp;&nbsp;&nbsp;5 |&nbsp;&nbsp;&nbsp;&nbsp;&nbsp;&nbsp;2 |&nbsp;&nbsp;&nbsp;Yes |&nbsp;&nbsp;green |<br>
      | | target 2 |&nbsp;&nbsp;&nbsp;&nbsp;20 |&nbsp;&nbsp;&nbsp;&nbsp;40 |&nbsp;&nbsp;&nbsp;red |&nbsp;&nbsp;&nbsp;&nbsp;10 |&nbsp;&nbsp;&nbsp;&nbsp;&nbsp;&nbsp;3 | Maybe | yellow |<br>
      | | target 3 |&nbsp;&nbsp;&nbsp;-40 |&nbsp;&nbsp;&nbsp;&nbsp;10 |&nbsp;&nbsp;blue |&nbsp;&nbsp;&nbsp;&nbsp;&nbsp;3 |&nbsp;&nbsp;&nbsp;&nbsp;&nbsp;&nbsp;4 | Wrong |&nbsp;&nbsp;&nbsp;&nbsp;red |
      | ----------------------------------------------------------------------<br>
      | 
      | 
      | </tt>
      | 
      | 
      | <p>Inputs:<br>
      | <B> Target_Row: </B> this scalar input determines which row in the Target Table is used to define the target parameters. Typically the Target_Row comes from the Trial_Protocol.  <P>
      | <B> Target_State: </B> this scalar input determines which state the target is in. Different states reference different columns in the Target Table (as defined in the Dialog Box). Typically the Target_State input is controlled by the Stateflow chart to dynamically change the appearance of the target depending on system and/or subject behavior. Target_State=0 is a valid input, which turns the target off. The intended method for turning a target off is to set Target_State=0. <BR>
      | <P>
      | <B>Opacity:</B> This input is only available if Source for Opacity is selected as port, in which case the opacity for all of the targets created by this block is specified as a percentage.
      | The length of this input must either match the length of the Target_Row(s) input (i.e. which case each Opacity maps to the appropriate Target_row)
      | or this input must be a scalar (in which case the Opacity maps to all of the Target_Rows).<BR>
      | <P>
      | There is one output from this block:
      | <P>
      | <B> VCODE: </B> this output is a vector containing one VCODE. This output must go to the Process_Video_CMD block of the video library for the target to actually be shown (if any other visual targets are to be displayed, then this VCODE output must be concatenated with the other VCODES prior to connection to the Process_Video_CMD block - see Help for the Process_Video_CMD block for more information).
      | <P>
      | To show multiple targets simultaneously, multiple copies of the Show_Target and Show_Target_With_Label blocks can be used in a Task Program. The output VCODES from multiple Show_Target and Show_Target_With_Label blocks must be concatenated prior to connection to the Process_Video_CMD block.
      | <P>
      | 
      | <H2>Parameters and Dialog Box</H2>
      | <B>Type of Target:</B> Choose the type of target specified in the target table.
      | <P>
      | <B>Number of Target States:</B> Choose the number of target states specified in each target row. Up to five target states are allowed per target row.
      | <P>
      | <B>State [n] Target Table Columns:</B> Enter the column indices that specify the relevant target attributes in the Target Table. All target types have the same first three target attributes (fill colour, stroke colour and stroke width) and the same last three target attributes (label text, label colour, and label height).
      | <Blockquote>
      | <P>
      | Element 1 (fill colour) - points to the column index in the Target Table containing the fill colour. If this index is 0, then the fill colour is transparent and the Target Table is not referenced. For line targets, the fill colour is not used.
      | <P>
      | Element 2 (stroke colour) - points to the column index in the Target Table containing the stroke colour. If this index is 0, then the stroke colour is transparent and the Target Table is not referenced. It is possible to use the same column index for both fill colour and stroke colour (i.e.  if single-colour targets are desired). For line targets, stroke colour defines the colour of the line.
      | <P>
      | Element 3 (stroke width) - points to the column index in the Target Table containing the stroke width (cm). If no stroke is desired, then setting the stroke column index to 0 will produce a stroke width of 0  and the Target Table is not referenced.  Setting stroke column index to a value less than 0 will produce a standard 1 mm stroke width, again without referencing the Target Table. For line targets, stroke width defines the width of the line.
      | <P>
      | <B><I>Circle</I></B> <P>
      | Element 4 (radius) - radius of the circle (cm).
      | <P>
      | <B><I>Ellipse</I></B> <P>
      | Elements 4-6 (ellipse properties) - major radius (cm), minor radius (cm), rotation angle (degrees). If no rotation is desired, then setting rotation column index to 0 will produce a default rotation of 0 and the Target Table will not be referenced.
      | <P>
      | <B><I>Rectangle</I></B><P>
      | Elements 4-6 (rectangle properties) - length (cm), height (cm), rotation angle (degrees). If no rotation is desired, then setting rotation column index to 0 will produce a default rotation of 0 and the Target Table will not be referenced.
      | <P>
      | <B><I>Line</I></B><P>
      | Elements 4-5 (line properties) - end point x-axis position relative to start point (cm), end point y-axis position relative to start point (cm). The width and colour of the line are defined by the stroke width and the stroke colour, respectively. The fill colour column is ignored (i.e. any value can be used for column 1)
      | <P>
      | <B><I>Triangle</I></B><P>
      | Elements 4-7 (triangle properties) - length (cm), height (cm), offset of peak of triangle relative to midpoint of the length (cm), rotation angle (degrees). If a height column index of 0 is specified, then an equilateral triangle with sides of the specified length will be created and the Target Table will not be referenced for height or peak offset. If no rotation is desired, then setting a rotation column index of 0 will produce a default rotation of 0 and the Target Table will not be referenced.
      | <P>
      | <B><I>Label</I></B>
      | <P>
      | The last three elements of the target state vector define the label. In order, these elements are:
      | <P>
      | Label text - the index of the column in the Target Table containing the text used for the label (up to 50 characters).
      | <P>
      | Label colour - the index of the column in the Target Table containing the label colour. If this index is 0, then the label colour is transparent and the Target Table is not referenced.
      | <P>
      | Label height - the index of the column in the Target Table containing the label height (cm).
      | </Blockquote>
      | <P>
      | Each target state requires its own set of column index definitions (although multiple states can point to the same column index if desired).<P>
      | 
      | <B>Source for Opacity:</B> Choose either dialog, to specify the opacity in this dialog, or port, which will create a new input to allow dynamic control of opacity.
      | <P>
      | <B>Opacity:</B> This parameter is only available if Source for Opacity is selected as dialog, in which case the opacity for all of the targets created by this block is specified as a percentage.
      | <P>
      | <B>Target Display:</B> This option determines whether the target(s) are shown on the operator display only, the subject display only, or both displays.
      | <P>
      | 
      | <H2>Examples</H2>
      | 
      | <B>Example 1:</B>  Suppose a target row will be used to define 1 state for an ellipse type target. It will be an outline of an ellipse with a label in the center (using a stroke colour and a standard 1mm stroke width). The related Target Table columns are:
      | <P>
      | column 4 = colour<BR>
      | column 5 = major radius<BR>
      | column 6 = minor radius<BR>
      | column 7 = orientation<BR>
      | column 8 = label text<BR>
      | column 9 = label colour<BR>
      | column 10 = label height
      | <P>For this example, "State 1 Target Table Columns" would equal [0 4 -1 5 6 7 8 9 10].
      | <P>
      | 
      | <H2>Related Blocks </H2>
      | Show_Target<BR>
      | Process_Video_CMD
      mask TypeOptions target_type: Circle | Ellipse | Rectangle | Line | Triangle
      mask Callback target_type:
      | %%%%
      | % Because of bugs iN R2007, R2010a and R2013a (which have been reported to Mathworks), the following code
      | % is required here because in the Initialization Section it will ONLY correctly update those Mask Parameters that are hidden
      | % when the OK button is clicked (NOTE: the initialization code will correctly update all Mask Parameters when the Apply button
      | % is clicked, the bug is that it should also update everything when the OK button is clicked in the absence of an Apply click)
      | %
      | % Adding a set_param call which updates one of the mask parameters will call the initialization code to run, which "avoids"
      | % this bug. This code should be removed once Mathworks has fixed this bug.
      | 
      | temp = get_param(gcb, 'target_type');
      | set_param(gcb, 'target_type', temp);
      mask TypeOptions num_states: 1 | 2 | 3 | 4 | 5
      mask Callback num_states:
      | block_path=gcb;
      | num_states=str2num(get_param(block_path, 'num_states'));
      | vis=get_param(block_path,'MaskVisibilities');
      | 
      | %If the number of states>1, then output an array instead of a vector.
      | %Only show those inputs necessary on the Mask
      | output_block=char(find_system(block_path,'LookUnderMasks','all','SearchDepth',1,'BlockType','Outport'));
      | if num_states==1			%output of HandInTarget block is a vector
      | 	vis{4}='off';
      | 	vis{5}='off';
      | 	vis{6}='off';
      | 	vis{7}='off';
      | elseif num_states==2					%output of HandInTarget block is an array
      | 	vis{4}='on';
      | 	vis{5}='off';
      | 	vis{6}='off';
      | 	vis{7}='off';
      | elseif num_states==3					%output of HandInTarget block is an array
      | 	vis{4}='on';
      | 	vis{5}='on';
      | 	vis{6}='off';
      | 	vis{7}='off';
      | elseif num_states==4					%output of HandInTarget block is an array
      | 	vis{4}='on';
      | 	vis{5}='on';
      | 	vis{6}='on';
      | 	vis{7}='off';
      | else								%output of HandInTarget block is an array
      | 	vis{4}='on';
      | 	vis{5}='on';
      | 	vis{6}='on';
      | 	vis{7}='on';
      | end
      | set_param(block_path,'MaskVisibilities',vis);
      mask TypeOptions source: dialog | port
      mask Callback source:
      | % Show or hide the opacity input on the mask dialog
      | sourceStr=get_param(gcb,'source');
      | vis=get_param(gcb,'MaskVisibilities');
      | 
      | if strmatch(sourceStr, 'dialog')
      | 	vis{10}='on';
      | else
      | 	vis{10}='off';
      | end
      | 
      | set_param(gcb,'MaskVisibilities',vis);
      mask TypeOptions target_display: Both subject and operator displays | Subject display only | Operator display only
      mask Display: disp(columntext); port_label('output',1,outputname); port_label('input',1, inputname1); port_label('input',2, inputname2);
  EMG Processing : Subsystem
  GUI Control : General/GUI Control  target_type_str=Circle  Target_Type=1  XYcols=[1 2]  Vcols=3  Lcols=4  indices_padding=[0 0 0 0;0 0 0 0]  task_version=1.0  show_repeat_trial_flag=off
  KINARM_Apply_Loads : KINARM_loads/KINARM_Apply_Loads  up_duration=1500  down_duration=1500  max_torque=10
  KINARM_EP_Apply_Loads : KINARM_EP_loads/KINARM_EP_Apply_Loads  up_duration=1500  down_duration=1500  max_force=60
  MATLAB Function : MATLAB Function  TreatAsAtomicUnit=on
  MATLAB Function1 : MATLAB Function  TreatAsAtomicUnit=on
  Matrix Concatenate : Concatenate  NumInputs=7  Mode=Multidimensional array
  Mux : Mux  Inputs=11
  Mux{1,3..7,9..10} (8 alike) : Mux  Inputs=2
  Mux2 : Mux  Inputs=3
  Mux8 : Mux  Inputs=16
  Pair 1 : xpclib/Misc./Scope (xPC)   Priority=4  scopeno=1  scopetype=Target  autostart=on  viewmode=Graphical rolling  formatstr='%15.6f'  grid=on  ylimits=[-1,1]  nosamples=1000  noprepostsamples=0  interleave=5  triggermode=FreeRun  triggersignal=1  trigsignalfromport=off  triggerlevel=0.0  triggerslope=Either  triggerscope=1  triggersample=0  filename=data.dat  mode=Lazy  writesize=512  autorestart=off  dynamicfilemode=off  maxwritefilesize=512*1024^2
  Pair 2 : xpclib/Misc./Scope (xPC)   Priority=4  scopeno=2  scopetype=Target  autostart=on  viewmode=Graphical rolling  formatstr='%15.6f'  grid=on  ylimits=[-1,1]  nosamples=1000  noprepostsamples=0  interleave=5  triggermode=FreeRun  triggersignal=1  trigsignalfromport=off  triggerlevel=0.0  triggerslope=Either  triggerscope=1  triggersample=0  filename=data.dat  mode=Lazy  writesize=512  autorestart=off  dynamicfilemode=off  maxwritefilesize=512*1024^2
  Pair 3 : xpclib/Misc./Scope (xPC)   Priority=4  scopeno=3  scopetype=Target  autostart=on  viewmode=Graphical rolling  formatstr='%15.6f'  grid=on  ylimits=[-1,1]  nosamples=1000  noprepostsamples=0  interleave=5  triggermode=FreeRun  triggersignal=1  trigsignalfromport=off  triggerlevel=0.0  triggerslope=Either  triggerscope=1  triggersample=0  filename=data.dat  mode=Lazy  writesize=512  autorestart=off  dynamicfilemode=off  maxwritefilesize=512*1024^2
  Pair 4 : xpclib/Misc./Scope (xPC)   Priority=4  scopeno=4  scopetype=Target  autostart=on  viewmode=Graphical rolling  formatstr='%15.6f'  grid=on  ylimits=[-1,1]  nosamples=1000  noprepostsamples=0  interleave=5  triggermode=FreeRun  triggersignal=1  trigsignalfromport=off  triggerlevel=0.0  triggerslope=Either  triggerscope=1  triggersample=0  filename=data.dat  mode=Lazy  writesize=512  autorestart=off  dynamicfilemode=off  maxwritefilesize=512*1024^2
  Pair 5 : xpclib/Misc./Scope (xPC)   Priority=4  scopeno=5  scopetype=Target  autostart=on  viewmode=Graphical rolling  formatstr='%15.6f'  grid=on  ylimits=[-1,1]  nosamples=1000  noprepostsamples=0  interleave=5  triggermode=FreeRun  triggersignal=1  trigsignalfromport=off  triggerlevel=0.0  triggerslope=Either  triggerscope=1  triggersample=0  filename=data.dat  mode=Lazy  writesize=512  autorestart=off  dynamicfilemode=off  maxwritefilesize=512*1024^2
  Pair 6 : xpclib/Misc./Scope (xPC)   Priority=4  scopeno=6  scopetype=Target  autostart=on  viewmode=Graphical rolling  formatstr='%15.6f'  grid=on  ylimits=[-1,1]  nosamples=1000  noprepostsamples=0  interleave=5  triggermode=FreeRun  triggersignal=1  trigsignalfromport=off  triggerlevel=0.0  triggerslope=Either  triggerscope=1  triggersample=0  filename=data.dat  mode=Lazy  writesize=512  autorestart=off  dynamicfilemode=off  maxwritefilesize=512*1024^2
  Pair 7 : xpclib/Misc./Scope (xPC)   Priority=4  scopeno=7  scopetype=Target  autostart=on  viewmode=Graphical rolling  formatstr='%15.6f'  grid=on  ylimits=[-1,1]  nosamples=1000  noprepostsamples=0  interleave=5  triggermode=FreeRun  triggersignal=1  trigsignalfromport=off  triggerlevel=0.0  triggerslope=Either  triggerscope=1  triggersample=0  filename=data.dat  mode=Lazy  writesize=512  autorestart=off  dynamicfilemode=off  maxwritefilesize=512*1024^2
  Pair 8 : xpclib/Misc./Scope (xPC)   Priority=4  scopeno=8  scopetype=Target  autostart=on  viewmode=Graphical rolling  formatstr='%15.6f'  grid=on  ylimits=[-1,1]  nosamples=1000  noprepostsamples=0  interleave=5  triggermode=FreeRun  triggersignal=1  trigsignalfromport=off  triggerlevel=0.0  triggerslope=Either  triggerscope=1  triggersample=0  filename=data.dat  mode=Lazy  writesize=512  autorestart=off  dynamicfilemode=off  maxwritefilesize=512*1024^2
  Pair 9 : xpclib/Misc./Scope (xPC)   Priority=4  scopeno=9  scopetype=Target  autostart=on  viewmode=Graphical rolling  formatstr='%15.6f'  grid=on  ylimits=[-1,1]  nosamples=1000  noprepostsamples=0  interleave=5  triggermode=FreeRun  triggersignal=1  trigsignalfromport=off  triggerlevel=0.0  triggerslope=Either  triggerscope=1  triggersample=0  filename=data.dat  mode=Lazy  writesize=512  autorestart=off  dynamicfilemode=off  maxwritefilesize=512*1024^2
  Parameter Table Defn : General/Parameter Table Defn  ShowInLibBrowser=0
  Parameter_columns : Subsystem  AncestorBlock=Video/Show_Target_With_Label  mask(Show_Target_With_Label){target_type=Circle, num_states=1, attribcol1=[START_X START_Y 0 0 TARGET_RADIUS 0 0], attribcol2=[6 6 0 3 0 0 0], attribcol3=[0 0 0 0 0 0 0], attribcol4=[0 0 0 0 0 0 0], attribcol5=[0 0 24 0 0 0 0], stateindices_padding=[0 0 0 0;0 0 0 0;0 0 0 0;0 0 0 0;0 0 0 0], source=dialog, opacity=100, target_display=Both subject and operator displays}
      mask prompts: target_type "Type of Target"; num_states "Number of Target States"; attribcol1 "State 1 Target Table Column(s)"; attribcol2 "State 2 Target Table Column(s)"; attribcol3 "State 3 Target Table Column(s)"; attribcol4 "State 4 Target Table Column(s)"; attribcol5 "State 5 Target Table Column(s)"; stateindices_padding "State Indices Padding"; source "Source for Opacity"; target_display "Target Display"
      mask help: This block returns a VCODE that, when sent to the Process_Video_CMD block, will cause a single target with a text label to be drawn. The label will be centered at the centroid of the target. Target parameters are specified in the Target Table according to the columns defined below and the row input to this block.
      mask init: same as BimanualCarvingModifiedOldEMG/Draw_Hand_Endpoint
      mask Help:
      | Used to draw a single, stationary target with a label.
      | 
      | <H2>Library </H2>
      | Video
      | 
      | <H2>Description </H2>
      | This block returns a VCODE, which when sent to the Process_Video_CMD block will draw a single stationary target with a label. The VCODE contains all of the target parameters necessary to draw the target and the label.
      | <P>
      | The VCODE is generated from information contained in the Target Table. Which parts of the Target Table are used is determined by the columns selected (see Parameters and Dialog Box below).<P>
      | 
      | <p>For example, assume the "row" input is 2, the "type of target" is set to "rectangle" and the "Target Table Columns" is set to [3 0 0 4 5 0 6 7 4].
      | Then using the sample target table below a red rectangle will be drawn at (20cm, 40cm) with a width of 10cm and a height of 3cm.
      | The rectangle will have the word "Maybe" in yellow on it in letters 3cm heigh. The zeros in the  "Target Table Columns" indicate those parameters are not used (i.e. no stroke color, no stroke width, and no rotation).
      | 
      | <p><tt>
      | ______________________________________________________________________<br>
      | |&nbsp;&nbsp;&nbsp;&nbsp;&nbsp;&nbsp;&nbsp;&nbsp;&nbsp;&nbsp;| X Pos | Y pos |&nbsp;&nbsp;Fill | Width | Height |&nbsp;&nbsp;Text | TColor |<br>
      | ----------------------------------------------------------------------<br>
      | | target 1 |&nbsp;&nbsp;&nbsp;&nbsp;10 |&nbsp;&nbsp;&nbsp;&nbsp;10 | white |&nbsp;&nbsp;&nbsp;&nbsp;&nbsp;5 |&nbsp;&nbsp;&nbsp;&nbsp;&nbsp;&nbsp;2 |&nbsp;&nbsp;&nbsp;Yes |&nbsp;&nbsp;green |<br>
      | | target 2 |&nbsp;&nbsp;&nbsp;&nbsp;20 |&nbsp;&nbsp;&nbsp;&nbsp;40 |&nbsp;&nbsp;&nbsp;red |&nbsp;&nbsp;&nbsp;&nbsp;10 |&nbsp;&nbsp;&nbsp;&nbsp;&nbsp;&nbsp;3 | Maybe | yellow |<br>
      | | target 3 |&nbsp;&nbsp;&nbsp;-40 |&nbsp;&nbsp;&nbsp;&nbsp;10 |&nbsp;&nbsp;blue |&nbsp;&nbsp;&nbsp;&nbsp;&nbsp;3 |&nbsp;&nbsp;&nbsp;&nbsp;&nbsp;&nbsp;4 | Wrong |&nbsp;&nbsp;&nbsp;&nbsp;red |
      | ----------------------------------------------------------------------<br>
      | 
      | 
      | </tt>
      | 
      | 
      | <p>Inputs:<br>
      | <B> Target_Row: </B> this scalar input determines which row in the Target Table is used to define the target parameters. Typically the Target_Row comes from the Trial_Protocol.  <P>
      | <B> Target_State: </B> this scalar input determines which state the target is in. Different states reference different columns in the Target Table (as defined in the Dialog Box). Typically the Target_State input is controlled by the Stateflow chart to dynamically change the appearance of the target depending on system and/or subject behavior. Target_State=0 is a valid input, which turns the target off. The intended method for turning a target off is to set Target_State=0. <BR>
      | <P>
      | <B>Opacity:</B> This input is only available if Source for Opacity is selected as port, in which case the opacity for all of the targets created by this block is specified as a percentage.
      | The length of this input must either match the length of the Target_Row(s) input (i.e. which case each Opacity maps to the appropriate Target_row)
      | or this input must be a scalar (in which case the Opacity maps to all of the Target_Rows).<BR>
      | <P>
      | There is one output from this block:
      | <P>
      | <B> VCODE: </B> this output is a vector containing one VCODE. This output must go to the Process_Video_CMD block of the video library for the target to actually be shown (if any other visual targets are to be displayed, then this VCODE output must be concatenated with the other VCODES prior to connection to the Process_Video_CMD block - see Help for the Process_Video_CMD block for more information).
      | <P>
      | To show multiple targets simultaneously, multiple copies of the Show_Target and Show_Target_With_Label blocks can be used in a Task Program. The output VCODES from multiple Show_Target and Show_Target_With_Label blocks must be concatenated prior to connection to the Process_Video_CMD block.
      | <P>
      | 
      | <H2>Parameters and Dialog Box</H2>
      | <B>Type of Target:</B> Choose the type of target specified in the target table.
      | <P>
      | <B>Number of Target States:</B> Choose the number of target states specified in each target row. Up to five target states are allowed per target row.
      | <P>
      | <B>State [n] Target Table Columns:</B> Enter the column indices that specify the relevant target attributes in the Target Table. All target types have the same first three target attributes (fill colour, stroke colour and stroke width) and the same last three target attributes (label text, label colour, and label height).
      | <Blockquote>
      | <P>
      | Element 1 (fill colour) - points to the column index in the Target Table containing the fill colour. If this index is 0, then the fill colour is transparent and the Target Table is not referenced. For line targets, the fill colour is not used.
      | <P>
      | Element 2 (stroke colour) - points to the column index in the Target Table containing the stroke colour. If this index is 0, then the stroke colour is transparent and the Target Table is not referenced. It is possible to use the same column index for both fill colour and stroke colour (i.e.  if single-colour targets are desired). For line targets, stroke colour defines the colour of the line.
      | <P>
      | Element 3 (stroke width) - points to the column index in the Target Table containing the stroke width (cm). If no stroke is desired, then setting the stroke column index to 0 will produce a stroke width of 0  and the Target Table is not referenced.  Setting stroke column index to a value less than 0 will produce a standard 1 mm stroke width, again without referencing the Target Table. For line targets, stroke width defines the width of the line.
      | <P>
      | <B><I>Circle</I></B> <P>
      | Element 4 (radius) - radius of the circle (cm).
      | <P>
      | <B><I>Ellipse</I></B> <P>
      | Elements 4-6 (ellipse properties) - major radius (cm), minor radius (cm), rotation angle (degrees). If no rotation is desired, then setting rotation column index to 0 will produce a default rotation of 0 and the Target Table will not be referenced.
      | <P>
      | <B><I>Rectangle</I></B><P>
      | Elements 4-6 (rectangle properties) - length (cm), height (cm), rotation angle (degrees). If no rotation is desired, then setting rotation column index to 0 will produce a default rotation of 0 and the Target Table will not be referenced.
      | <P>
      | <B><I>Line</I></B><P>
      | Elements 4-5 (line properties) - end point x-axis position relative to start point (cm), end point y-axis position relative to start point (cm). The width and colour of the line are defined by the stroke width and the stroke colour, respectively. The fill colour column is ignored (i.e. any value can be used for column 1)
      | <P>
      | <B><I>Triangle</I></B><P>
      | Elements 4-7 (triangle properties) - length (cm), height (cm), offset of peak of triangle relative to midpoint of the length (cm), rotation angle (degrees). If a height column index of 0 is specified, then an equilateral triangle with sides of the specified length will be created and the Target Table will not be referenced for height or peak offset. If no rotation is desired, then setting a rotation column index of 0 will produce a default rotation of 0 and the Target Table will not be referenced.
      | <P>
      | <B><I>Label</I></B>
      | <P>
      | The last three elements of the target state vector define the label. In order, these elements are:
      | <P>
      | Label text - the index of the column in the Target Table containing the text used for the label (up to 50 characters).
      | <P>
      | Label colour - the index of the column in the Target Table containing the label colour. If this index is 0, then the label colour is transparent and the Target Table is not referenced.
      | <P>
      | Label height - the index of the column in the Target Table containing the label height (cm).
      | </Blockquote>
      | <P>
      | Each target state requires its own set of column index definitions (although multiple states can point to the same column index if desired).<P>
      | 
      | <B>Source for Opacity:</B> Choose either dialog, to specify the opacity in this dialog, or port, which will create a new input to allow dynamic control of opacity.
      | <P>
      | <B>Opacity:</B> This parameter is only available if Source for Opacity is selected as dialog, in which case the opacity for all of the targets created by this block is specified as a percentage.
      | <P>
      | <B>Target Display:</B> This option determines whether the target(s) are shown on the operator display only, the subject display only, or both displays.
      | <P>
      | 
      | <H2>Examples</H2>
      | 
      | <B>Example 1:</B>  Suppose a target row will be used to define 1 state for an ellipse type target. It will be an outline of an ellipse with a label in the center (using a stroke colour and a standard 1mm stroke width). The related Target Table columns are:
      | <P>
      | column 4 = colour<BR>
      | column 5 = major radius<BR>
      | column 6 = minor radius<BR>
      | column 7 = orientation<BR>
      | column 8 = label text<BR>
      | column 9 = label colour<BR>
      | column 10 = label height
      | <P>For this example, "State 1 Target Table Columns" would equal [0 4 -1 5 6 7 8 9 10].
      | <P>
      | 
      | <H2>Related Blocks </H2>
      | Show_Target<BR>
      | Process_Video_CMD
      mask TypeOptions target_type: Circle | Ellipse | Rectangle | Line | Triangle
      mask Callback target_type:
      | %%%%
      | % Because of bugs iN R2007, R2010a and R2013a (which have been reported to Mathworks), the following code
      | % is required here because in the Initialization Section it will ONLY correctly update those Mask Parameters that are hidden
      | % when the OK button is clicked (NOTE: the initialization code will correctly update all Mask Parameters when the Apply button
      | % is clicked, the bug is that it should also update everything when the OK button is clicked in the absence of an Apply click)
      | %
      | % Adding a set_param call which updates one of the mask parameters will call the initialization code to run, which "avoids"
      | % this bug. This code should be removed once Mathworks has fixed this bug.
      | 
      | temp = get_param(gcb, 'target_type');
      | set_param(gcb, 'target_type', temp);
      mask TypeOptions num_states: 1 | 2 | 3 | 4 | 5
      mask Callback num_states:
      | block_path=gcb;
      | num_states=str2num(get_param(block_path, 'num_states'));
      | vis=get_param(block_path,'MaskVisibilities');
      | 
      | %If the number of states>1, then output an array instead of a vector.
      | %Only show those inputs necessary on the Mask
      | output_block=char(find_system(block_path,'LookUnderMasks','all','SearchDepth',1,'BlockType','Outport'));
      | if num_states==1			%output of HandInTarget block is a vector
      | 	vis{4}='off';
      | 	vis{5}='off';
      | 	vis{6}='off';
      | 	vis{7}='off';
      | elseif num_states==2					%output of HandInTarget block is an array
      | 	vis{4}='on';
      | 	vis{5}='off';
      | 	vis{6}='off';
      | 	vis{7}='off';
      | elseif num_states==3					%output of HandInTarget block is an array
      | 	vis{4}='on';
      | 	vis{5}='on';
      | 	vis{6}='off';
      | 	vis{7}='off';
      | elseif num_states==4					%output of HandInTarget block is an array
      | 	vis{4}='on';
      | 	vis{5}='on';
      | 	vis{6}='on';
      | 	vis{7}='off';
      | else								%output of HandInTarget block is an array
      | 	vis{4}='on';
      | 	vis{5}='on';
      | 	vis{6}='on';
      | 	vis{7}='on';
      | end
      | set_param(block_path,'MaskVisibilities',vis);
      mask TypeOptions source: dialog | port
      mask Callback source:
      | % Show or hide the opacity input on the mask dialog
      | sourceStr=get_param(gcb,'source');
      | vis=get_param(gcb,'MaskVisibilities');
      | 
      | if strmatch(sourceStr, 'dialog')
      | 	vis{10}='on';
      | else
      | 	vis{10}='off';
      | end
      | 
      | set_param(gcb,'MaskVisibilities',vis);
      mask TypeOptions target_display: Both subject and operator displays | Subject display only | Operator display only
      mask Display: disp(columntext); port_label('output',1,outputname); port_label('input',1, inputname1); port_label('input',2, inputname2);
  Process_Video_CMD : Video/Process_Video_CMD
  Selector1 : Selector  NumberOfDimensions=2  InputPortWidth=3  IndexOptions=Select all,Starting index (port)  Indices=[1 3],1  OutputSizes=1,1
  Selector{3..4,6..7,9..11,17} (8 alike) : Selector  NumberOfDimensions=2  InputPortWidth=1  IndexOptions=Select all,Starting index (port)  Indices=[1 3],1  OutputSizes=1,1
  Selector2 : Selector  NumberOfDimensions=2  InputPortWidth=3  IndexOptions=Index vector (port),Select all  Indices=[1 3],1  OutputSizes=1,1
  Selector5 : Selector  NumberOfDimensions=2  InputPortWidth=3  IndexOptions=Select all,Starting index (port)  Indices=[1 3],1  OutputSizes=1,1
  Selector8 : Selector  NumberOfDimensions=2  InputPortWidth=3  IndexOptions=Select all,Starting index (port)  Indices=[1 3],1  OutputSizes=1,1
  Show_Target_With_Label : Video/Show_Target_With_Label  target_type=Rectangle  num_states=1  attribcol1=[TEXT_COLOR 0 0 TEXTBOX_WIDTH TEXTBOX_HEIGHT ROTATION LABEL_TEXT LABEL_COLOR LABEL_HEIGHT]  attribcol2=[6 6 0 3 0 0 0 0 0]  attribcol3=[0 0 0 0 0 0 0 0 0]  attribcol4=[0 0 0 0 0 0 0 0 0]  attribcol5=[0 0 24 0 0 0 0 0 0]  stateindices_padding=[0 0;0 0;0 0;0 0;0 0]  source=dialog  opacity=100  target_display=Both subject and operator displays
  Trajectory subsystem : Subsystem
  Trial_Control : Stateflow chart  TreatAsAtomicUnit=on
  emgScoreVCode : MATLAB Function  TreatAsAtomicUnit=on
  function : MATLAB Function  TreatAsAtomicUnit=on
  sample_buffer : MATLAB Function  TreatAsAtomicUnit=on
  Constant : Constant  IOType=siggen
  tag scope: ForceOn=global, HandDistance=global, HandVelXL=global, HandVelXR=global, HandVelYL=global, HandVelYR=global, MaterialDamping=global, MaterialDuctility=global, MaterialMass=global, MaterialPos=global, MaterialTargetPos=global, MaterialUpdateInd1=global, MaterialUpdateInd2=global, R2Score=global, ScaleVibration=global, StoneWidth=global, emgBuffer=global, event_code=global, kHands=global, kMaterial=global, materialPosY=global, maxEMG_on=global, minEMG_on=global, normalizeEMG_on=global, processedEMG=global, rawSignal=global, residualBuffer=global, smoothnessScore=global, trial_state=global, xForceRobotL=global, xForceRobotR=global, xStart=global, yFinish=global, yForceRobotL=global, yForceRobotR=global, yStart=global, yWall=global
  wires:
  Trial_Control/1(logging_enable) -> DataLogging/1
  Trial_Control/9(e_Trial_End) -> GUI Control/1
  Trajectory subsystem/2(EXO Torques) -> KINARM_Apply_Loads/1
  Trajectory subsystem/1(EP forces) -> KINARM_EP_Apply_Loads/1
  Constant4/1 -> Parameter_columns/2(Target_State)
  Draw_Hand_Endpoint/1(VCODE) -> Trajectory subsystem/2(target_position), Matrix Concatenate/1
  MATLAB Function1/1(HandAtStart) -> Trial_Control/2(HandAtStart)
  Trial_Control/2(trial_state) -> [trial_state], Mux/1
  Mux/1 -> DataLogging/3
  Matrix Concatenate/1 -> Process_Video_CMD/1
  Trial_Control/3(ForceOn) -> [ForceOn]
  Constant5/1 -> Selector1/2
  Selector1/1 -> Parameter_columns/1(Target_Row)
  Constant6/1 -> Trajectory subsystem/1(Duration)
  Draw_Start/1(VCODE) -> Matrix Concatenate/2
  Selector5/1 -> Selector2/2
  [Load_Table] -> Selector2/1
  Selector2/1 -> Selector9/1, Selector7/1, Selector6/1, Selector4/1, Selector3/1, Selector17/1
  MATLAB Function1/3(xStart) -> [xStart]
  MATLAB Function1/4(yStart) -> [yStart]
  [trial_state] -> function/2(trial_state)
  Constant2/1 -> Selector17/2
  Selector17/1 -> [kMaterial]
  [KINdata] -> function/1(KINdata)
  function/1(MaterialPos) -> [MaterialPos]
  Constant3/1 -> Selector3/2
  Selector3/1 -> [MaterialMass]
  [kMaterial] -> function/3(kMaterial)
  [MaterialMass] -> function/4(MaterialMass)
  function/3(MaterialUpdateInd1) -> [MaterialUpdateInd1]
  function/4(MaterialUpdateInd2) -> [MaterialUpdateInd2]
  Constant8/1 -> Selector4/2
  Selector4/1 -> [MaterialDamping]
  [MaterialDamping] -> function/5(MaterialDamping)
  [yStart] -> function/7(yStart)
  Constant7/1 -> Selector5/2
  Mux5/1 -> Pair 3/1
  Mux6/1 -> Pair 4/1
  Mux7/1 -> Pair 5/1
  [xStart] -> function/6(xStart)
  function/5(xForceRobotL) -> [xForceRobotL]
  function/6(yForceRobotL) -> [yForceRobotL]
  MATLAB Function1/5(HandVelXR) -> [HandVelXR]
  MATLAB Function1/6(HandVelYR) -> [HandVelYR]
  MATLAB Function1/7(HandVelXL) -> [HandVelXL]
  MATLAB Function1/8(HandVelYL) -> [HandVelYL]
  [HandVelXR] -> Mux/2
  [HandVelYR] -> Mux/3
  [HandVelXL] -> Mux/4
  [HandVelYL] -> Mux/5
  [HandDistance] -> function/8(HandDistance)
  Constant12/1 -> Selector6/2
  Selector6/1 -> [kHands]
  [kHands] -> function/9(kHands)
  Draw_Material/1(VCODE) -> Matrix Concatenate/5
  function/7(xForceRobotR) -> [xForceRobotR]
  function/8(yForceRobotR) -> [yForceRobotR]
  Draw_target/1(VCODE) -> Matrix Concatenate/3
  function/9(yWall) -> [yWall]
  Draw_MaterialTarget/1(VCODE) -> Matrix Concatenate/4
  function/2(MaterialTargetPos) -> [MaterialTargetPos]
  [ScaleVibration] -> function/10(ScaleVibration)
  Constant13/1 -> Selector7/2
  Selector7/1 -> [ScaleVibration]
  Draw_finish_line/1(VCODE) -> Matrix Concatenate/6
  MATLAB Function1/10(yFinish) -> [yFinish]
  MATLAB Function1/2(HandAtFinish) -> Trial_Control/3(HandAtFinish)
  GUI Control/2 -> Trial_Control/1(Trial_Protocol), Selector5/1, Selector1/1, Selector8/1
  Constant14/1 -> Selector8/2
  Selector8/1 -> [StoneWidth]
  [StoneWidth] -> function/11(stoneWidth)
  Selector9/1 -> [MaterialDuctility]
  Constant16/1 -> Selector9/2
  [MaterialDuctility] -> function/12(materialDuctility)
  [processedEMG] -> MATLAB Function/1(emg)
  Constant1/1 -> Draw_Start/2(Target_State), Draw_target/1(Target_Row), Draw_target/2(Target_State), Draw_MaterialTarget/1(Target_Row), Draw_MaterialTarget/2(Target_State), Show_Target_With_Label/2, Show_Target_With_Label/1, Draw_finish_line/2(Target_State), Draw_finish_line/1(Target_Row), Draw_message/2(Target_State), Draw_message/1(Target_Row), Draw_Material/2(Target_State), Draw_Material/1(Target_Row), Draw_Start/1(Target_Row), Draw_Hand_Endpoint/1(Target_Row), Draw_Hand_Endpoint/2(Target_State)
  Show_Target_With_Label/1 -> emgScoreVCode/1(VCODE)
  [emgBuffer] -> emgScoreVCode/2(emgBuffer)
  sample_buffer/1(res_history) -> [residualBuffer]
  sample_buffer/2(d_history) -> [emgBuffer]
  [residualBuffer] -> emgScoreVCode/3(residualBuffer)
  MATLAB Function/1(resid) -> sample_buffer/1(resid_sample)
  [MaterialUpdateInd1] -> Mux/6
  [MaterialUpdateInd2] -> Mux/7
  [rawSignal] -> Bus Selector/1
  Bus Selector/1 -> Mux3/1  "<signal1>"
  Bus Selector/2 -> Mux3/2  "<signal2>"
  [rawSignal] -> Bus Selector1/1
  Bus Selector1/1 -> Mux4/1  "<signal3>"
  Bus Selector1/2 -> Mux4/2  "<signal4>"
  [rawSignal] -> Bus Selector2/1
  Bus Selector2/1 -> Mux5/1  "<signal5>"
  Bus Selector2/2 -> Mux5/2  "<signal6>"
  [rawSignal] -> Bus Selector3/1
  Bus Selector3/1 -> Mux6/1  "<signal7>"
  Bus Selector3/2 -> Mux6/2  "<signal8>"
  [rawSignal] -> Bus Selector4/1
  Bus Selector4/1 -> Mux7/1  "<signal9>"
  Bus Selector4/2 -> Mux7/2  "<signal10>"
  [rawSignal] -> Bus Selector5/1
  Bus Selector5/1 -> Mux1/1  "<signal11>"
  Bus Selector5/2 -> Mux1/2  "<signal12>"
  [rawSignal] -> Mux/10
  [rawSignal] -> EMG Processing/1(In1)
  EMG Processing/1(Out1) -> Pair 9/1, [processedEMG]
  [task_control_button] -> Compare To Constant/1
  GUI Control/1 -> Mux2/1
  Compare To Constant/1 -> Mux2/2
  Mux2/1 -> Trial_Control/Trigger
  [task_control_button] -> Compare To Constant1/1
  Compare To Constant1/1 -> Mux2/3
  Trial_Control/6(maxEMG_on) -> [maxEMG_on]
  [maxEMG_on] -> EMG Processing/3(In3)
  Trial_Control/7(normalizeEMG_on) -> [normalizeEMG_on]
  [normalizeEMG_on] -> EMG Processing/4(In4)
  Trial_Control/8(event_code) -> [event_code]
  [event_code] -> DataLogging/2
  Trial_Control/5(minEMG_on) -> [minEMG_on]
  [minEMG_on] -> EMG Processing/2(In2)
  Analog Inputs1/1 -> Mux8/1
  Analog Inputs1/2 -> Mux8/2
  Analog Inputs1/3 -> Mux8/3
  Analog Inputs1/4 -> Mux8/4
  Analog Inputs1/5 -> Mux8/5
  Analog Inputs1/6 -> Mux8/6
  Analog Inputs1/7 -> Mux8/7
  Analog Inputs1/8 -> Mux8/8
  Analog Inputs1/9 -> Mux8/9
  Analog Inputs1/10 -> Mux8/10
  Analog Inputs1/11 -> Mux8/11
  Analog Inputs1/12 -> Mux8/12
  Analog Inputs1/13 -> Mux8/13
  Analog Inputs1/14 -> Mux8/14
  Analog Inputs1/15 -> Mux8/15
  Analog Inputs1/16 -> Mux8/16
  Mux8/1 -> [rawSignal]
  Mux3/1 -> Pair 1/1
  Mux4/1 -> Pair 2/1
  Mux1/1 -> Pair 6/1
  Mux10/1 -> Pair 7/1
  [rawSignal] -> Bus Selector6/1
  Bus Selector6/2 -> Mux10/1  "<signal14>"
  Bus Selector6/1 -> Mux10/2  "<signal13>"
  [rawSignal] -> Bus Selector7/1
  Bus Selector7/1 -> Mux9/1  "<signal15>"
  Bus Selector7/2 -> Mux9/2  "<signal16>"
  Mux9/1 -> Pair 8/1
  [processedEMG] -> sample_buffer/2(d_sample)
  emgScoreVCode/1(VCODE_out) -> Matrix Concatenate/7
  MATLAB Function1/9(HandDistance) -> [HandDistance]
  [Task_Wide_Parameters] -> Selector10/1
  Constant9/1 -> Selector10/2
  Selector10/1 -> MATLAB Function/2(syn_num)
  [Task_Wide_Parameters] -> Selector11/1
  Constant10/1 -> Selector11/2
  Selector11/1 -> MATLAB Function1/3(hand_distance)
  Parameter_columns/1(VCODE) -> MATLAB Function1/1(SET_EXP_PARAMS1)
  [KINdata] -> MATLAB Function1/2(KINdata)
  emgScoreVCode/2(R2) -> [R2Score]
  [R2Score] -> Mux/8
  [smoothnessScore] -> Mux/9
  function/11(smoothnessScore) -> [smoothnessScore]
  [smoothnessScore] -> emgScoreVCode/4(smoothnessScore)
  function/10(materialPosY) -> [materialPosY]
  [materialPosY] -> Mux/11
